simulink model "normal"  (R2020a)
settings: Solver=ode45  StartTime=0.0  StopTime=0.4  FixedStep=1e-6  MaxStep=0.04  RelTol=1e-3  EnableMultiTasking=on
PreLoadFcn:
  | power_13NodeTestFeeder_init;
values from neighbouring files (symbols this model uses):
  C_601 = [1.03835973183e-08  -3.28956213337e-09  -2.07596127216e-09; -3.28956213337e-09  9.8230300863e-09  -1.22250137004e-09; -2.07596127216e-09  -1.22250137004e-09  9.29377945947e-09]    [Finalmat.mat]    (also in bus1.mat; bus10.mat; bus11.mat; bus12.mat)
  C_602 = [9.39333329896e-09  -1.78290377777e-09  -2.78635373607e-09; -1.78290377777e-09  8.5370713848e-09  -1.08586207709e-09; -2.78635373607e-09  -1.08586207709e-09  8.94105559107e-09]    [Finalmat.mat]    (also in bus1.mat; bus10.mat; bus11.mat; bus12.mat)
  C_603 = [0  0  0; 0  7.76272711671e-09  -1.48325331387e-09; 0  -1.48325331387e-09  7.69036927641e-09]    [Finalmat.mat]    (also in bus1.mat; bus10.mat; bus11.mat; bus12.mat)
  C_604 = [7.69036927641e-09  0  -1.48325331387e-09; 0  0  0; -1.48325331387e-09  0  7.76272711671e-09]    [Finalmat.mat]    (also in bus1.mat; bus10.mat; bus11.mat; bus12.mat)
  C_605 = [0  0  0; 0  0  0; 0  0  7.44890176838e-09]    [Finalmat.mat]    (also in bus1.mat; bus10.mat; bus11.mat; bus12.mat)
  C_606 = [1.59697709306e-07  -1.64824237567e-15  -1.64824237567e-15; -1.64824237567e-15  1.59697709306e-07  -1.64824237567e-15; -1.64824237567e-15  -1.64824237567e-15  1.59697709306e-07]    [Finalmat.mat]    (also in bus1.mat; bus10.mat; bus11.mat; bus12.mat)
  C_607 = [1.46679066902e-07  0  0; 0  0  0; 0  0  0]    [Finalmat.mat]    (also in bus1.mat; bus10.mat; bus11.mat; bus12.mat)
  ft2km = 0.0003048    [Finalmat.mat]    (also in bus1.mat; bus10.mat; bus11.mat; bus12.mat)
  L_601 = [0.0016777459142  0.000826923199875  0.000698195470335; 0.000826923199875  0.00172702836123  0.000634408490396; 0.000698195470335  0.000634408490396  0.00170560121035]    [Finalmat.mat]    (also in bus1.mat; bus10.mat; bus11.mat; bus12.mat)
  L_602 = [0.00194723354262  0.000698195470335  0.000826923199875; 0.000698195470335  0.00197508883877  0.000634408490396; 0.000826923199875  0.000634408490396  0.00199635116541]    [Finalmat.mat]    (also in bus1.mat; bus10.mat; bus11.mat; bus12.mat)
  L_603 = [0  0  0; 0  0.00222034730427  0.000756708074671; 0  0.000756708074671  0.00223650007955]    [Finalmat.mat]    (also in bus1.mat; bus10.mat; bus11.mat; bus12.mat)
  L_604 = [0.00223650007955  0  0.000756708074671; 0  0  0; 0.000756708074671  0  0.00222034730427]    [Finalmat.mat]    (also in bus1.mat; bus10.mat; bus11.mat; bus12.mat)
  L_605 = [0  0  0; 0  0  0; 0  0  0.00222100660122]    [Finalmat.mat]    (also in bus1.mat; bus10.mat; bus11.mat; bus12.mat)
  L_606 = [0.000735610572263  5.40623499221e-05  2.35698659721e-05; 5.40623499221e-05  0.000666054744009  5.40623499221e-05; 2.35698659721e-05  5.40623499221e-05  0.000735610572263]    [Finalmat.mat]    (also in bus1.mat; bus10.mat; bus11.mat; bus12.mat)
  L_607 = [0.000844559393295  0  0; 0  0  0; 0  0  0]    [Finalmat.mat]    (also in bus1.mat; bus10.mat; bus11.mat; bus12.mat)
  R_601 = [0.215305653249  0.0969341469174  0.0981768923907; 0.0969341469174  0.209713298619  0.0953807150757; 0.0981768923907  0.0953807150757  0.212136652292]    [Finalmat.mat]    (also in bus1.mat; bus10.mat; bus11.mat; bus12.mat)
  R_602 = [0.467645121603  0.0981768923907  0.0969341469174; 0.0981768923907  0.464476120646  0.0953807150757; 0.0969341469174  0.0953807150757  0.462052766973]    [Finalmat.mat]    (also in bus1.mat; bus10.mat; bus11.mat; bus12.mat)
  R_603 = [0  0  0; 0  0.826052916102  0.128375607392; 0  0.128375607392  0.822573228777]    [Finalmat.mat]    (also in bus1.mat; bus10.mat; bus11.mat; bus12.mat)
  R_604 = [0.822573228777  0  0.128375607392; 0  0  0; 0.128375607392  0  0.826052916102]    [Finalmat.mat]    (also in bus1.mat; bus10.mat; bus11.mat; bus12.mat)
  R_605 = [0  0  0; 0  0  0; 0  0  0.825928641555]    [Finalmat.mat]    (also in bus1.mat; bus10.mat; bus11.mat; bus12.mat)
  R_606 = [0.495979718394  0.198342177539  0.177029092672; 0.198342177539  0.49032522649  0.198342177539; 0.177029092672  0.198342177539  0.495979718394]    [Finalmat.mat]    (also in bus1.mat; bus10.mat; bus11.mat; bus12.mat)
  R_607 = [0.834192898952  0  0; 0  0  0; 0  0  0]    [Finalmat.mat]    (also in bus1.mat; bus10.mat; bus11.mat; bus12.mat)
libraries: neural x322, powerlib x54, powerlib_meascontrol x6, simulink x1
(part 5 of 8)

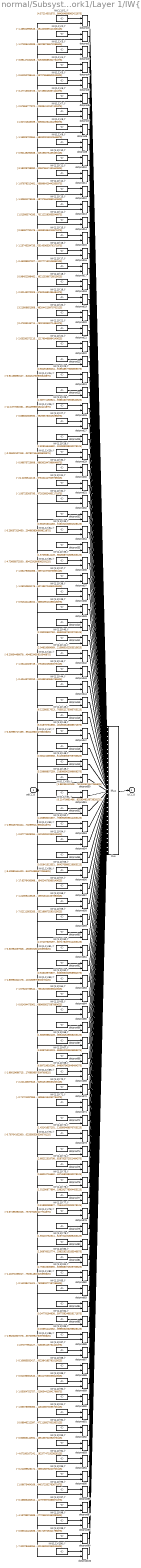
== system normal/Subsystem1/Function Fitting Neural Network1/Layer 1/IW{1,1} ==
  "pd{1,1}" : Inport  PortDimensions=9
      mask Display: e = 0.06;c1 = [120 230 180]/255;c2 = ([120 230 180]+0)/(256+128);c3 = ([120 230 180]+128)/(256+128);patch([0 1 1 0],[0 0 1 1],c1);patch([0 1 1 1-e 1-e 0+e],[0 0 1 1-e 0+e 0+e],c2);patch([0 0 1 1-e 0+e 0+e],[0 1 1 1-e 1-e 0+e],c3);plot([0 1 1 0 0],[0 0 1 1 0]);
  "IW{1,1}(1,:)'" : Constant  Value=[4.57214501575121357035413893754594027996063232421875;1.882606225958038503875968672218732535839080810546875;-5.8020031488986969492316347896121442317962646484375;-1.893288066425211635390724040917120873928070068359375;-0.8587623785139932852672473018174059689044952392578125;4.75157469500696638675663052708841860294342041015625;-8.5282617700155807227702098316513001918792724609375;-3.382695445647363907681892669643275439739227294921875;5.878872822846187062850731308571994304656982421875]
      mask Display: e = 0.06;c1 = [120 150 230]/255;c2 = ([120 150 230]+0)/383;c3 = ([120 150 230]+128)/383;patch([0 1 1 0],[0 0 1 1],c1);patch([0 1 1 1-e 1-e 0+e],[0 0 1 1-e 0+e 0+e],c2);patch([0 0 1 1-e 0+e 0+e],[0 1 1 1-e 1-e 0+e],c3);plot([0 1 1 0 0],[0 0 1 1 0]);disp('Weights');
  "IW{1,1}(10,:)'" : Constant  Value=[-0.901492906386826664544287268654443323612213134765625;-0.113174797714675090531954992911778390407562255859375;1.080394196679439033914604806341230869293212890625;-0.73545756418224861317156637596781365573406219482421875;-0.5017931218574249729869052316644228994846343994140625;-1.384370210252817923191059890086762607097625732421875;0.142477760614644177739052111064665950834751129150390625;0.047994454507014831790012721057792077772319316864013671875;-1.07906134729644254122149504837580025196075439453125]
      mask Display: e = 0.06;c1 = [120 150 230]/255;c2 = ([120 150 230]+0)/383;c3 = ([120 150 230]+128)/383;patch([0 1 1 0],[0 0 1 1],c1);patch([0 1 1 1-e 1-e 0+e],[0 0 1 1-e 0+e 0+e],c2);patch([0 0 1 1-e 0+e 0+e],[0 1 1 1-e 1-e 0+e],c3);plot([0 1 1 0 0],[0 0 1 1 0]);disp('Weights');
  "IW{1,1}(100,:)'" : Constant  Value=[-7.320784632640833677896807785145938396453857421875;-16.1707657106398841051486670039594173431396484375;7.2803217921115379596130878780968487262725830078125;3.3426274799199280352013374795205891132354736328125;2.874821735640806341649522437364794313907623291015625;4.61847119975394004853797014220617711544036865234375;1.3255014486968230702501614359789527952671051025390625;0.304284782798684094728969284915365278720855712890625;-0.269542146930250636760462157326401211321353912353515625]
      mask Display: e = 0.06;c1 = [120 150 230]/255;c2 = ([120 150 230]+0)/383;c3 = ([120 150 230]+128)/383;patch([0 1 1 0],[0 0 1 1],c1);patch([0 1 1 1-e 1-e 0+e],[0 0 1 1-e 0+e 0+e],c2);patch([0 0 1 1-e 0+e 0+e],[0 1 1 1-e 1-e 0+e],c3);plot([0 1 1 0 0],[0 0 1 1 0]);disp('Weights');
  "IW{1,1}(11,:)'" : Constant  Value=[3.182097989903924339927243636338971555233001708984375;-1.2350123444631406766092140969703905284404754638671875;2.388405963368278595027049959753639996051788330078125;-0.86926885397664677146423173326184041798114776611328125;-1.060735410466756345471139866276644170284271240234375;-0.2099496708397343980312399480681051500141620635986328125;4.97375374438937267740357128786854445934295654296875;0.59049268116716879806205042768851853907108306884765625;1.0899488888556165822052435032674111425876617431640625]
      mask Display: e = 0.06;c1 = [120 150 230]/255;c2 = ([120 150 230]+0)/383;c3 = ([120 150 230]+128)/383;patch([0 1 1 0],[0 0 1 1],c1);patch([0 1 1 1-e 1-e 0+e],[0 0 1 1-e 0+e 0+e],c2);patch([0 0 1 1-e 0+e 0+e],[0 1 1 1-e 1-e 0+e],c3);plot([0 1 1 0 0],[0 0 1 1 0]);disp('Weights');
  "IW{1,1}(12,:)'" : Constant  Value=[-1.8787831248148643137341196052148006856441497802734375;0.8158366697060552841236358290188945829868316650390625;1.8402745283322923253166436552419327199459075927734375;-2.500087171504715488623560304404236376285552978515625;0.6981167220195245715075316184083931148052215576171875;0.68711892811027308614058028979343362152576446533203125;-2.837133552361146282549952957197092473506927490234375;2.6394050270587587903037274372763931751251220703125;2.250006537446691989856617510668002068996429443359375]
      mask Display: e = 0.06;c1 = [120 150 230]/255;c2 = ([120 150 230]+0)/383;c3 = ([120 150 230]+128)/383;patch([0 1 1 0],[0 0 1 1],c1);patch([0 1 1 1-e 1-e 0+e],[0 0 1 1-e 0+e 0+e],c2);patch([0 0 1 1-e 0+e 0+e],[0 1 1 1-e 1-e 0+e],c3);plot([0 1 1 0 0],[0 0 1 1 0]);disp('Weights');
  "IW{1,1}(13,:)'" : Constant  Value=[-1.30581276345382235604120069183409214019775390625;-0.0578981895339648333642657007658272050321102142333984375;-0.200199831873287881212064576175180263817310333251953125;0.32696800181646079597186371756833977997303009033203125;0.51819519715458894904003273040871135890483856201171875;-1.05830517304619053930991867673583328723907470703125;-0.90740435735102398240314869326539337635040283203125;-0.428920341006585770227133025400689803063869476318359375;-0.53095640707807023606079610544838942587375640869140625]
      mask Display: e = 0.06;c1 = [120 150 230]/255;c2 = ([120 150 230]+0)/383;c3 = ([120 150 230]+128)/383;patch([0 1 1 0],[0 0 1 1],c1);patch([0 1 1 1-e 1-e 0+e],[0 0 1 1-e 0+e 0+e],c2);patch([0 0 1 1-e 0+e 0+e],[0 1 1 1-e 1-e 0+e],c3);plot([0 1 1 0 0],[0 0 1 1 0]);disp('Weights');
  "IW{1,1}(14,:)'" : Constant  Value=[1.5158057429565598983600693827611394226551055908203125;-1.53943291617461053277793325833044946193695068359375;1.1719124189160725624248016174533404409885406494140625;0.91568727726024423674289209884591400623321533203125;-0.91349144230285539425295837645535357296466827392578125;0.129574899846442492812315094852237962186336517333984375;1.357529536973298700530676796915940940380096435546875;0.9917911601413254008008379969396628439426422119140625;-0.53992566084737869669396559402230195701122283935546875]
      mask Display: e = 0.06;c1 = [120 150 230]/255;c2 = ([120 150 230]+0)/383;c3 = ([120 150 230]+128)/383;patch([0 1 1 0],[0 0 1 1],c1);patch([0 1 1 1-e 1-e 0+e],[0 0 1 1-e 0+e 0+e],c2);patch([0 0 1 1-e 0+e 0+e],[0 1 1 1-e 1-e 0+e],c3);plot([0 1 1 0 0],[0 0 1 1 0]);disp('Weights');
  "IW{1,1}(15,:)'" : Constant  Value=[0.3636779247682031535049418380367569625377655029296875;0.27580226552316544630372163737774826586246490478515625;0.91847507041818976514235828290111385285854339599609375;0.94676222259045050844150637203711085021495819091796875;1.1914278164934548609465991830802522599697113037109375;1.0862301664903963871466885393601842224597930908203125;-0.313351448219361838898322503155213780701160430908203125;0.480054965682457090991874792962335050106048583984375;-1.0512469187967610206868585009942762553691864013671875]
      mask Display: e = 0.06;c1 = [120 150 230]/255;c2 = ([120 150 230]+0)/383;c3 = ([120 150 230]+128)/383;patch([0 1 1 0],[0 0 1 1],c1);patch([0 1 1 1-e 1-e 0+e],[0 0 1 1-e 0+e 0+e],c2);patch([0 0 1 1-e 0+e 0+e],[0 1 1 1-e 1-e 0+e],c3);plot([0 1 1 0 0],[0 0 1 1 0]);disp('Weights');
  "IW{1,1}(16,:)'" : Constant  Value=[-1.2374533473535482830385490160551853477954864501953125;0.84525543133610880897066408579121343791484832763671875;-1.1637539518642545655069397980696521699428558349609375;0.2051190480644304037216585356873110868036746978759765625;2.659058217179519179040880771935917437076568603515625;0.2220786361148645859930894630451803095638751983642578125;0.256689466162800361548335104089346714317798614501953125;0.32918163162337654714661994148627854883670806884765625;-1.539386232767935069887244026176631450653076171875]
      mask Display: e = 0.06;c1 = [120 150 230]/255;c2 = ([120 150 230]+0)/383;c3 = ([120 150 230]+128)/383;patch([0 1 1 0],[0 0 1 1],c1);patch([0 1 1 1-e 1-e 0+e],[0 0 1 1-e 0+e 0+e],c2);patch([0 0 1 1-e 0+e 0+e],[0 1 1 1-e 1-e 0+e],c3);plot([0 1 1 0 0],[0 0 1 1 0]);disp('Weights');
  "IW{1,1}(17,:)'" : Constant  Value=[-0.4528993702754127159693098292336799204349517822265625;0.2996485110712263644217046021367423236370086669921875;-1.3571742827353954208291497707250528037548065185546875;0.72201368049507952395771326337126083672046661376953125;-0.260676388954095783478948078482062555849552154541015625;-1.7370101028329736347899370230152271687984466552734375;-0.72478751750280301369144808631972409784793853759765625;1.6961692464966287019478841102682054042816162109375;-2.777268542019787123109608728555031120777130126953125]
      mask Display: e = 0.06;c1 = [120 150 230]/255;c2 = ([120 150 230]+0)/383;c3 = ([120 150 230]+128)/383;patch([0 1 1 0],[0 0 1 1],c1);patch([0 1 1 1-e 1-e 0+e],[0 0 1 1-e 0+e 0+e],c2);patch([0 0 1 1-e 0+e 0+e],[0 1 1 1-e 1-e 0+e],c3);plot([0 1 1 0 0],[0 0 1 1 0]);disp('Weights');
  "IW{1,1}(18,:)'" : Constant  Value=[0.984523984828047371564707646030001342296600341796875;0.440886294126075828359034858294762670993804931640625;-0.6759076310964935441205625465954653918743133544921875;-1.289035500093658637155158430687151849269866943359375;-0.7106270365609741457291193000855855643749237060546875;-0.00059208655953670529491217333628583219251595437526702880859375;2.360279246169174616198915828135795891284942626953125;2.289325113655392041067671016207896173000335693359375;0.61338355224400320508948425413109362125396728515625]
      mask Display: e = 0.06;c1 = [120 150 230]/255;c2 = ([120 150 230]+0)/383;c3 = ([120 150 230]+128)/383;patch([0 1 1 0],[0 0 1 1],c1);patch([0 1 1 1-e 1-e 0+e],[0 0 1 1-e 0+e 0+e],c2);patch([0 0 1 1-e 0+e 0+e],[0 1 1 1-e 1-e 0+e],c3);plot([0 1 1 0 0],[0 0 1 1 0]);disp('Weights');
  "IW{1,1}(19,:)'" : Constant  Value=[-2.32143070023364384013575545395724475383758544921875;1.35427998731956922284780375775881111621856689453125;-1.1460257544519387717940617221756838262081146240234375;-0.5807263512829130558401402595336548984050750732421875;1.0079516669472294854159599708509631454944610595703125;-2.12978652832783499349034173064865171909332275390625;0.6223670523531816822782047893269918859004974365234375;-1.4856321514957333551620877187815494835376739501953125;0.04807060918235782354113183600929914973676204681396484375]
      mask Display: e = 0.06;c1 = [120 150 230]/255;c2 = ([120 150 230]+0)/383;c3 = ([120 150 230]+128)/383;patch([0 1 1 0],[0 0 1 1],c1);patch([0 1 1 1-e 1-e 0+e],[0 0 1 1-e 0+e 0+e],c2);patch([0 0 1 1-e 0+e 0+e],[0 1 1 1-e 1-e 0+e],c3);plot([0 1 1 0 0],[0 0 1 1 0]);disp('Weights');
  "IW{1,1}(2,:)'" : Constant  Value=[-1.465049905469430147064713310101069509983062744140625;-0.1874316016641332238723549608039320446550846099853515625;-0.06919763970673868669347683635351131670176982879638671875;-0.57055203810173826806106944786733947694301605224609375;3.1381492483832875706184495356865227222442626953125;-0.874421368308234026045511200209148228168487548828125;1.23739151157753735077449164236895740032196044921875;1.3521956808911073100176736261346377432346343994140625;4.10697081729739910116450118948705494403839111328125]
      mask Display: e = 0.06;c1 = [120 150 230]/255;c2 = ([120 150 230]+0)/383;c3 = ([120 150 230]+128)/383;patch([0 1 1 0],[0 0 1 1],c1);patch([0 1 1 1-e 1-e 0+e],[0 0 1 1-e 0+e 0+e],c2);patch([0 0 1 1-e 0+e 0+e],[0 1 1 1-e 1-e 0+e],c3);plot([0 1 1 0 0],[0 0 1 1 0]);disp('Weights');
  "IW{1,1}(20,:)'" : Constant  Value=[3.218086519585205973470465323771350085735321044921875;-16.27590168275634852079747361131012439727783203125;17.987410545814295659283743589185178279876708984375;3.758242055086093547089376443182118237018585205078125;-4.85910970919836326942231607972644269466400146484375;0.3725222076867311660208770263125188648700714111328125;-1.3744616444228034968233487234101630747318267822265625;-5.007581197173916365272816619835793972015380859375;0.24849610765830132397269380817306227982044219970703125]
      mask Display: e = 0.06;c1 = [120 150 230]/255;c2 = ([120 150 230]+0)/383;c3 = ([120 150 230]+128)/383;patch([0 1 1 0],[0 0 1 1],c1);patch([0 1 1 1-e 1-e 0+e],[0 0 1 1-e 0+e 0+e],c2);patch([0 0 1 1-e 0+e 0+e],[0 1 1 1-e 1-e 0+e],c3);plot([0 1 1 0 0],[0 0 1 1 0]);disp('Weights');
  "IW{1,1}(21,:)'" : Constant  Value=[0.47333245711844529335365905353683046996593475341796875;-6.1031253338012145803759267437271773815155029296875;2.142440438103456745722041887347586452960968017578125;2.62530251915655110650504866498522460460662841796875;-1.841367984976616245518243886181153357028961181640625;1.9183672712002162175082276007742621004581451416015625;1.1140395667070130958364870821242220699787139892578125;-0.09091837053477576369164836478375946171581745147705078125;0.8327519583244809009414666434167884290218353271484375]
      mask Display: e = 0.06;c1 = [120 150 230]/255;c2 = ([120 150 230]+0)/383;c3 = ([120 150 230]+128)/383;patch([0 1 1 0],[0 0 1 1],c1);patch([0 1 1 1-e 1-e 0+e],[0 0 1 1-e 0+e 0+e],c2);patch([0 0 1 1-e 0+e 0+e],[0 1 1 1-e 1-e 0+e],c3);plot([0 1 1 0 0],[0 0 1 1 0]);disp('Weights');
  "IW{1,1}(22,:)'" : Constant  Value=[-2.633303721159426569187189670628868043422698974609375;0.2855957397414907728006028264644555747509002685546875;-3.671941916130708083443323630490340292453765869140625;-0.70809683746574425544650921438005752861499786376953125;-0.83203434928004094128795031792833469808101654052734375;0.21652040710604414375239912260440178215503692626953125;-0.6855160542714191507229770650155842304229736328125;-0.77678134128400044833284709966392256319522857666015625;-0.465629395082590991084003917421796359121799468994140625]
      mask Display: e = 0.06;c1 = [120 150 230]/255;c2 = ([120 150 230]+0)/383;c3 = ([120 150 230]+128)/383;patch([0 1 1 0],[0 0 1 1],c1);patch([0 1 1 1-e 1-e 0+e],[0 0 1 1-e 0+e 0+e],c2);patch([0 0 1 1-e 0+e 0+e],[0 1 1 1-e 1-e 0+e],c3);plot([0 1 1 0 0],[0 0 1 1 0]);disp('Weights');
  "IW{1,1}(23,:)'" : Constant  Value=[0.56491806234007679865527506990474648773670196533203125;0.77026935261504358987139085002127103507518768310546875;-0.064774393859191981004386207132483832538127899169921875;1.849415015758316460647847634390927851200103759765625;0.96274697549558718723261563354753889143466949462890625;-1.1368993403818092868817757334909401834011077880859375;0.86488128146804121865187653384055010974407196044921875;0.351346425363474157421705967863090336322784423828125;-0.425453238706487935072431127991876564919948577880859375]
      mask Display: e = 0.06;c1 = [120 150 230]/255;c2 = ([120 150 230]+0)/383;c3 = ([120 150 230]+128)/383;patch([0 1 1 0],[0 0 1 1],c1);patch([0 1 1 1-e 1-e 0+e],[0 0 1 1-e 0+e 0+e],c2);patch([0 0 1 1-e 0+e 0+e],[0 1 1 1-e 1-e 0+e],c3);plot([0 1 1 0 0],[0 0 1 1 0]);disp('Weights');
  "IW{1,1}(24,:)'" : Constant  Value=[-0.91138890127663374496336246011196635663509368896484375;15.0789832454367029868080862797796726226806640625;10.556078107952632905153222964145243167877197265625;-0.9792542115477893549524424088303931057453155517578125;3.0303379951251638857456782716326415538787841796875;-2.761581601481574832490650805993936955928802490234375;-8.3770890674707967349377213395200669765472412109375;-2.070123180109808114224279051995836198329925537109375;-13.6068544965806932367513581993989646434783935546875]
      mask Display: e = 0.06;c1 = [120 150 230]/255;c2 = ([120 150 230]+0)/383;c3 = ([120 150 230]+128)/383;patch([0 1 1 0],[0 0 1 1],c1);patch([0 1 1 1-e 1-e 0+e],[0 0 1 1-e 0+e 0+e],c2);patch([0 0 1 1-e 0+e 0+e],[0 1 1 1-e 1-e 0+e],c3);plot([0 1 1 0 0],[0 0 1 1 0]);disp('Weights');
  "IW{1,1}(25,:)'" : Constant  Value=[2.38771156921450966592601616866886615753173828125;-2.191485976358347187442632275633513927459716796875;3.00359378776327989868377699167467653751373291015625;-0.23173797831026388127639847880345769226551055908203125;-0.99380085545549778913709815242327749729156494140625;0.36246471125366774845844020092044956982135772705078125;2.794875124789037545980363574926741421222686767578125;-0.1950511468235609502386296298936940729618072509765625;-2.01187767968755171210659682401455938816070556640625]
      mask Display: e = 0.06;c1 = [120 150 230]/255;c2 = ([120 150 230]+0)/383;c3 = ([120 150 230]+128)/383;patch([0 1 1 0],[0 0 1 1],c1);patch([0 1 1 1-e 1-e 0+e],[0 0 1 1-e 0+e 0+e],c2);patch([0 0 1 1-e 0+e 0+e],[0 1 1 1-e 1-e 0+e],c3);plot([0 1 1 0 0],[0 0 1 1 0]);disp('Weights');
  "IW{1,1}(26,:)'" : Constant  Value=[-12.1377651561355168752243116614408791065216064453125;8.1591652697612939704185919254086911678314208984375;-3.80045548821983825149573021917603909969329833984375;-2.145339820153546295244950670166872441768646240234375;-3.71648549095900992966789999627508223056793212890625;6.57426106015730749021486190031282603740692138671875;4.48441260631393134872269001789391040802001953125;3.304872366104713687917637798818759620189666748046875;0.8970116797606457748059938239748589694499969482421875]
      mask Display: e = 0.06;c1 = [120 150 230]/255;c2 = ([120 150 230]+0)/383;c3 = ([120 150 230]+128)/383;patch([0 1 1 0],[0 0 1 1],c1);patch([0 1 1 1-e 1-e 0+e],[0 0 1 1-e 0+e 0+e],c2);patch([0 0 1 1-e 0+e 0+e],[0 1 1 1-e 1-e 0+e],c3);plot([0 1 1 0 0],[0 0 1 1 0]);disp('Weights');
  "IW{1,1}(27,:)'" : Constant  Value=[-0.88832363930812319186003378490568138659000396728515625;0.42785830611103670140238364183460362255573272705078125;0.80867323101893229253533945666276849806308746337890625;-0.77923766081130063643200855949544347822666168212890625;-0.56145456173519547871109125480870716273784637451171875;-0.60230053309847331188819907765719108283519744873046875;-1.3050830682250218472972846939228475093841552734375;-0.806330916403047215368360411957837641239166259765625;-0.441184745456177640487993585338699631392955780029296875]
      mask Display: e = 0.06;c1 = [120 150 230]/255;c2 = ([120 150 230]+0)/383;c3 = ([120 150 230]+128)/383;patch([0 1 1 0],[0 0 1 1],c1);patch([0 1 1 1-e 1-e 0+e],[0 0 1 1-e 0+e 0+e],c2);patch([0 0 1 1-e 0+e 0+e],[0 1 1 1-e 1-e 0+e],c3);plot([0 1 1 0 0],[0 0 1 1 0]);disp('Weights');
  "IW{1,1}(28,:)'" : Constant  Value=[2.82816646582525788033990465919487178325653076171875;0.35954363621026186326190554609638638794422149658203125;1.632878770180271832401786014088429510593414306640625;-0.0101763750096381978826887149125468567945063114166259765625;-1.059871357865847851797980183619074523448944091796875;-1.537916378610710399499339473550207912921905517578125;-0.316755007210310746135206727558397687971591949462890625;0.01847910556224353906262791724657290615141391754150390625;-2.461970474843802936248948753927834331989288330078125]
      mask Display: e = 0.06;c1 = [120 150 230]/255;c2 = ([120 150 230]+0)/383;c3 = ([120 150 230]+128)/383;patch([0 1 1 0],[0 0 1 1],c1);patch([0 1 1 1-e 1-e 0+e],[0 0 1 1-e 0+e 0+e],c2);patch([0 0 1 1-e 0+e 0+e],[0 1 1 1-e 1-e 0+e],c3);plot([0 1 1 0 0],[0 0 1 1 0]);disp('Weights');
  "IW{1,1}(29,:)'" : Constant  Value=[-0.2562310731830372834139097903971560299396514892578125;-0.026650997824419812853857791878908756189048290252685546875;0.5146222044853010491038958207354880869388580322265625;-0.08863109829785020821191210416145622730255126953125;1.0860301622782368990982604373130016028881072998046875;-0.83558626518929435267324379310593940317630767822265625;0.75271604021013638341486284843995235860347747802734375;-1.5471971637303971736088215038762427866458892822265625;-1.534789360688019854705999023281037807464599609375]
      mask Display: e = 0.06;c1 = [120 150 230]/255;c2 = ([120 150 230]+0)/383;c3 = ([120 150 230]+128)/383;patch([0 1 1 0],[0 0 1 1],c1);patch([0 1 1 1-e 1-e 0+e],[0 0 1 1-e 0+e 0+e],c2);patch([0 0 1 1-e 0+e 0+e],[0 1 1 1-e 1-e 0+e],c3);plot([0 1 1 0 0],[0 0 1 1 0]);disp('Weights');
  "IW{1,1}(3,:)'" : Constant  Value=[-1.273064109391197629150838110945187509059906005859375;-0.1746139127475550001378223896608687937259674072265625;-1.97988528255410134448766257264651358127593994140625;2.115356814135119112307847899501211941242218017578125;3.676111139990880349870394638855941593647003173828125;-0.634748668186627451603953886660747230052947998046875;-2.02947200057094079284070176072418689727783203125;0.70475348178681518351851309489575214684009552001953125;4.35348031629683962506760508404113352298736572265625]
      mask Display: e = 0.06;c1 = [120 150 230]/255;c2 = ([120 150 230]+0)/383;c3 = ([120 150 230]+128)/383;patch([0 1 1 0],[0 0 1 1],c1);patch([0 1 1 1-e 1-e 0+e],[0 0 1 1-e 0+e 0+e],c2);patch([0 0 1 1-e 0+e 0+e],[0 1 1 1-e 1-e 0+e],c3);plot([0 1 1 0 0],[0 0 1 1 0]);disp('Weights');
  "IW{1,1}(30,:)'" : Constant  Value=[-0.9987572360844405583435445805662311613559722900390625;-0.298860431335690790444203912556986324489116668701171875;-1.0756527117942642490788784925825893878936767578125;-0.2325361948543681334111710157230845652520656585693359375;-0.97740459386404177077878330237581394612789154052734375;0.1938044318657854148124641824324498884379863739013671875;0.8947266366516830604638244039961136877536773681640625;-0.6522406157472897536564460096997208893299102783203125;-1.1122828714271715266903584051760844886302947998046875]
      mask Display: e = 0.06;c1 = [120 150 230]/255;c2 = ([120 150 230]+0)/383;c3 = ([120 150 230]+128)/383;patch([0 1 1 0],[0 0 1 1],c1);patch([0 1 1 1-e 1-e 0+e],[0 0 1 1-e 0+e 0+e],c2);patch([0 0 1 1-e 0+e 0+e],[0 1 1 1-e 1-e 0+e],c3);plot([0 1 1 0 0],[0 0 1 1 0]);disp('Weights');
  "IW{1,1}(31,:)'" : Constant  Value=[-21.2230544116653589981069671921432018280029296875;17.38640835398523876165199908427894115447998046875;4.29589166719302806285440965439192950725555419921875;1.18972370473984323524518913473002612590789794921875;-1.649465861026556012802757322788238525390625;-1.4940892099984635077447592266253195703029632568359375;1.65452073013394596046055085025727748870849609375;-7.5067697997629547757014734088443219661712646484375;6.34941966304106841789689497090876102447509765625]
      mask Display: e = 0.06;c1 = [120 150 230]/255;c2 = ([120 150 230]+0)/383;c3 = ([120 150 230]+128)/383;patch([0 1 1 0],[0 0 1 1],c1);patch([0 1 1 1-e 1-e 0+e],[0 0 1 1-e 0+e 0+e],c2);patch([0 0 1 1-e 0+e 0+e],[0 1 1 1-e 1-e 0+e],c3);plot([0 1 1 0 0],[0 0 1 1 0]);disp('Weights');
  "IW{1,1}(32,:)'" : Constant  Value=[-1.9372530579534597006130525187472812831401824951171875;-0.034387366226837280669403895672076032496988773345947265625;-1.8460191297376915553485332566197030246257781982421875;-1.1491734164584344046744490697165019810199737548828125;-1.0773258382449684145143464775173924863338470458984375;0.5971848864048723282138553258846513926982879638671875;-1.0895137852805845124493089315365068614482879638671875;0.5721940530226146126580033524078316986560821533203125;-0.84712647433286036857680301181972026824951171875]
      mask Display: e = 0.06;c1 = [120 150 230]/255;c2 = ([120 150 230]+0)/383;c3 = ([120 150 230]+128)/383;patch([0 1 1 0],[0 0 1 1],c1);patch([0 1 1 1-e 1-e 0+e],[0 0 1 1-e 0+e 0+e],c2);patch([0 0 1 1-e 0+e 0+e],[0 1 1 1-e 1-e 0+e],c3);plot([0 1 1 0 0],[0 0 1 1 0]);disp('Weights');
  "IW{1,1}(33,:)'" : Constant  Value=[0.6529160448325892485144095189752988517284393310546875;-1.0012486019936506220773253517108969390392303466796875;0.404005214638427478934801229115691967308521270751953125;-0.08869602104426006772275314915532362647354602813720703125;1.5234337610562678211323373034247197210788726806640625;-0.0296601631566312147481045968788748723454773426055908203125;1.578527371192719019887817921699024736881256103515625;-0.483526252419098245827200344137963838875293731689453125;2.691032424683868828907407078077085316181182861328125]
      mask Display: e = 0.06;c1 = [120 150 230]/255;c2 = ([120 150 230]+0)/383;c3 = ([120 150 230]+128)/383;patch([0 1 1 0],[0 0 1 1],c1);patch([0 1 1 1-e 1-e 0+e],[0 0 1 1-e 0+e 0+e],c2);patch([0 0 1 1-e 0+e 0+e],[0 1 1 1-e 1-e 0+e],c3);plot([0 1 1 0 0],[0 0 1 1 0]);disp('Weights');
  "IW{1,1}(34,:)'" : Constant  Value=[-0.280373194502217704116020513538387604057788848876953125;-2.8648874605944225635312250233255326747894287109375;0.13981534693347297260146433472982607781887054443359375;-0.87154104232599227675137854021159000694751739501953125;0.59615182479228423506611989068915136158466339111328125;1.1000011216169645056339732036576606333255767822265625;-1.551372378155303710656198745709843933582305908203125;-2.730637946961703921289199570310302078723907470703125;-0.96224054502257139187548773406888358294963836669921875]
      mask Display: e = 0.06;c1 = [120 150 230]/255;c2 = ([120 150 230]+0)/383;c3 = ([120 150 230]+128)/383;patch([0 1 1 0],[0 0 1 1],c1);patch([0 1 1 1-e 1-e 0+e],[0 0 1 1-e 0+e 0+e],c2);patch([0 0 1 1-e 0+e 0+e],[0 1 1 1-e 1-e 0+e],c3);plot([0 1 1 0 0],[0 0 1 1 0]);disp('Weights');
  "IW{1,1}(35,:)'" : Constant  Value=[1.5709081414954437772024675723514519631862640380859375;-4.22386531174724577653023516177199780941009521484375;3.332881064917796010149686480872333049774169921875;-0.78210339536838191509815487734158523380756378173828125;0.43417624969241419563559247762896120548248291015625;1.200110893873937545350827349466271698474884033203125;-0.65289554267587568414654697335208766162395477294921875;5.60910565954152229295459619606845080852508544921875;-6.69035045844220821464887194451875984668731689453125]
      mask Display: e = 0.06;c1 = [120 150 230]/255;c2 = ([120 150 230]+0)/383;c3 = ([120 150 230]+128)/383;patch([0 1 1 0],[0 0 1 1],c1);patch([0 1 1 1-e 1-e 0+e],[0 0 1 1-e 0+e 0+e],c2);patch([0 0 1 1-e 0+e 0+e],[0 1 1 1-e 1-e 0+e],c3);plot([0 1 1 0 0],[0 0 1 1 0]);disp('Weights');
  "IW{1,1}(36,:)'" : Constant  Value=[-4.73608573200478932818668909021653234958648681640625;3.259068429729173654862961484468542039394378662109375;1.870367688521361149156518877134658396244049072265625;-3.9085077606485043588691041804850101470947265625;-0.132532681312490241420931624816148541867733001708984375;1.07321546901653075423155314638279378414154052734375;3.14899895426178577650944134802557528018951416015625;-1.0490359730371248137004158706986345350742340087890625;-5.4847780930769847174133246880955994129180908203125]
      mask Display: e = 0.06;c1 = [120 150 230]/255;c2 = ([120 150 230]+0)/383;c3 = ([120 150 230]+128)/383;patch([0 1 1 0],[0 0 1 1],c1);patch([0 1 1 1-e 1-e 0+e],[0 0 1 1-e 0+e 0+e],c2);patch([0 0 1 1-e 0+e 0+e],[0 1 1 1-e 1-e 0+e],c3);plot([0 1 1 0 0],[0 0 1 1 0]);disp('Weights');
  "IW{1,1}(37,:)'" : Constant  Value=[-1.6547906206673328455281080096028745174407958984375;-3.792463282037272787050596889457665383815765380859375;1.022480990224386321330030114040710031986236572265625;-1.41514034474598560109370737336575984954833984375;-0.0481143329803337127525963978769141249358654022216796875;-0.61324450181596523723470681943581439554691314697265625;-1.3073911340950215009826251844060607254505157470703125;-0.6260849341527563449716353716212324798107147216796875;-0.84798662852783213139673534897156059741973876953125]
      mask Display: e = 0.06;c1 = [120 150 230]/255;c2 = ([120 150 230]+0)/383;c3 = ([120 150 230]+128)/383;patch([0 1 1 0],[0 0 1 1],c1);patch([0 1 1 1-e 1-e 0+e],[0 0 1 1-e 0+e 0+e],c2);patch([0 0 1 1-e 0+e 0+e],[0 1 1 1-e 1-e 0+e],c3);plot([0 1 1 0 0],[0 0 1 1 0]);disp('Weights');
  "IW{1,1}(38,:)'" : Constant  Value=[-1.260105811766427219566821804619394242763519287109375;-0.86726445474906288524152842001058161258697509765625;4.4408342530586164542683036415837705135345458984375;5.05462080690503956503789595444686710834503173828125;-0.7458114846798424846241459817974828183650970458984375;-0.385168955880710262018595813060528598725795745849609375;-3.5337239758800560451845740317367017269134521484375;-4.59283664819310377680494639207608997821807861328125;-0.554578244091102678936522352159954607486724853515625]
      mask Display: e = 0.06;c1 = [120 150 230]/255;c2 = ([120 150 230]+0)/383;c3 = ([120 150 230]+128)/383;patch([0 1 1 0],[0 0 1 1],c1);patch([0 1 1 1-e 1-e 0+e],[0 0 1 1-e 0+e 0+e],c2);patch([0 0 1 1-e 0+e 0+e],[0 1 1 1-e 1-e 0+e],c3);plot([0 1 1 0 0],[0 0 1 1 0]);disp('Weights');
  "IW{1,1}(39,:)'" : Constant  Value=[-0.91342448152657784721242251180228777229785919189453125;-0.2276880613276453801940846233264892362058162689208984375;0.216120568324401018944769248264492489397525787353515625;0.279050464407995857385458293720148503780364990234375;-1.2470189329715950510291122554917819797992706298828125;-0.1573403547029812443724949844181537628173828125;-2.848487435814683887969067654921673238277435302734375;-1.501075399926252718074692893424071371555328369140625;-0.3034357923850758975703456599148921668529510498046875]
      mask Display: e = 0.06;c1 = [120 150 230]/255;c2 = ([120 150 230]+0)/383;c3 = ([120 150 230]+128)/383;patch([0 1 1 0],[0 0 1 1],c1);patch([0 1 1 1-e 1-e 0+e],[0 0 1 1-e 0+e 0+e],c2);patch([0 0 1 1-e 0+e 0+e],[0 1 1 1-e 1-e 0+e],c3);plot([0 1 1 0 0],[0 0 1 1 0]);disp('Weights');
  "IW{1,1}(4,:)'" : Constant  Value=[-3.89147184328426920529864219133742153644561767578125;3.459343926073256358932894727331586182117462158203125;-3.901582530636779733157482041860930621623992919921875;-1.2529766928303931461385900547611527144908905029296875;1.2930662567929680495382172011886723339557647705078125;-1.4188815690276730396846005533006973564624786376953125;3.30385499606749188927778959623537957668304443359375;4.30601828701230271434496899018995463848114013671875;-2.019042118362074145210272035910747945308685302734375]
      mask Display: e = 0.06;c1 = [120 150 230]/255;c2 = ([120 150 230]+0)/383;c3 = ([120 150 230]+128)/383;patch([0 1 1 0],[0 0 1 1],c1);patch([0 1 1 1-e 1-e 0+e],[0 0 1 1-e 0+e 0+e],c2);patch([0 0 1 1-e 0+e 0+e],[0 1 1 1-e 1-e 0+e],c3);plot([0 1 1 0 0],[0 0 1 1 0]);disp('Weights');
  "IW{1,1}(40,:)'" : Constant  Value=[2.280006327502011487240451970137655735015869140625;-2.960340871458381428737993701361119747161865234375;3.710286991107662135647160539519973099231719970703125;1.7881861683726614220546480282791890203952789306640625;-1.21956172031550824641499275458045303821563720703125;-0.61482727497653610893024733741185627877712249755859375;-3.215466035704943603690253439708612859249114990234375;0.390531736822932351582693399905110709369182586669921875;0.485190019842106690095562271380913443863391876220703125]
      mask Display: e = 0.06;c1 = [120 150 230]/255;c2 = ([120 150 230]+0)/383;c3 = ([120 150 230]+128)/383;patch([0 1 1 0],[0 0 1 1],c1);patch([0 1 1 1-e 1-e 0+e],[0 0 1 1-e 0+e 0+e],c2);patch([0 0 1 1-e 0+e 0+e],[0 1 1 1-e 1-e 0+e],c3);plot([0 1 1 0 0],[0 0 1 1 0]);disp('Weights');
  "IW{1,1}(41,:)'" : Constant  Value=[2.0481956906964580156227384577505290508270263671875;0.859554384584698905058530726819299161434173583984375;2.725886455265848606899226069799624383449554443359375;0.2260825309211777212059502062402316369116306304931640625;-0.82525102251196147395972957383492030203342437744140625;0.743435449833508510408819347503595054149627685546875;1.0238058376692169559873946127481758594512939453125;0.354984915450379967527538838112377561628818511962890625;-0.407063535495426676025232382016838528215885162353515625]
      mask Display: e = 0.06;c1 = [120 150 230]/255;c2 = ([120 150 230]+0)/383;c3 = ([120 150 230]+128)/383;patch([0 1 1 0],[0 0 1 1],c1);patch([0 1 1 1-e 1-e 0+e],[0 0 1 1-e 0+e 0+e],c2);patch([0 0 1 1-e 0+e 0+e],[0 1 1 1-e 1-e 0+e],c3);plot([0 1 1 0 0],[0 0 1 1 0]);disp('Weights');
  "IW{1,1}(42,:)'" : Constant  Value=[-6.2093446667831297958173308870755136013031005859375;-7.79394615880087204828896574326790869235992431640625;-0.233526348447979315015032852898002602159976959228515625;3.78428251311718089056057579000480473041534423828125;1.514861585424735590521549966069869697093963623046875;3.648175482940148928179269205429591238498687744140625;4.27427579049037742464633993222378194332122802734375;3.12509590011777493856470755417831242084503173828125;-1.145192992502511497576733745518140494823455810546875]
      mask Display: e = 0.06;c1 = [120 150 230]/255;c2 = ([120 150 230]+0)/383;c3 = ([120 150 230]+128)/383;patch([0 1 1 0],[0 0 1 1],c1);patch([0 1 1 1-e 1-e 0+e],[0 0 1 1-e 0+e 0+e],c2);patch([0 0 1 1-e 0+e 0+e],[0 1 1 1-e 1-e 0+e],c3);plot([0 1 1 0 0],[0 0 1 1 0]);disp('Weights');
  "IW{1,1}(43,:)'" : Constant  Value=[-1.33442026749275033381536559318192303180694580078125;-1.612620029591127046586507276515476405620574951171875;-0.34146945435227415988066468344186432659626007080078125;2.5259282671398981534593985998071730136871337890625;0.75062032032171488449279195265262387692928314208984375;3.183842110728863250557196806767024099826812744140625;3.505507379330950801232802405138500034809112548828125;2.21396331769093723806918205809779465198516845703125;5.14033135835540111457930834149010479450225830078125]
      mask Display: e = 0.06;c1 = [120 150 230]/255;c2 = ([120 150 230]+0)/383;c3 = ([120 150 230]+128)/383;patch([0 1 1 0],[0 0 1 1],c1);patch([0 1 1 1-e 1-e 0+e],[0 0 1 1-e 0+e 0+e],c2);patch([0 0 1 1-e 0+e 0+e],[0 1 1 1-e 1-e 0+e],c3);plot([0 1 1 0 0],[0 0 1 1 0]);disp('Weights');
  "IW{1,1}(44,:)'" : Constant  Value=[-0.404437320102107644714806156116537749767303466796875;-0.89483480675924198521897778846323490142822265625;-0.36393634805201580117994808460935018956661224365234375;-0.80784461164074772288046233370550908148288726806640625;-1.319887663125455024015764138312079012393951416015625;-0.517405527398214104550788761116564273834228515625;-2.619917563217764477911941867205314338207244873046875;-0.65019839853435268395287494058720767498016357421875;-5.38242466892981585857569371000863611698150634765625]
      mask Display: e = 0.06;c1 = [120 150 230]/255;c2 = ([120 150 230]+0)/383;c3 = ([120 150 230]+128)/383;patch([0 1 1 0],[0 0 1 1],c1);patch([0 1 1 1-e 1-e 0+e],[0 0 1 1-e 0+e 0+e],c2);patch([0 0 1 1-e 0+e 0+e],[0 1 1 1-e 1-e 0+e],c3);plot([0 1 1 0 0],[0 0 1 1 0]);disp('Weights');
  "IW{1,1}(45,:)'" : Constant  Value=[6.12288317013641947283986155525781214237213134765625;10.6304077127000482505536638200283050537109375;16.828317110034088699421772616915404796600341796875;0.480006240364688363531087134106201119720935821533203125;-3.030836669137740191359853270114399492740631103515625;-6.999151186851662487242720089852809906005859375;-5.9702070757160310421340909670107066631317138671875;-4.3988675496288056621096984599716961383819580078125;-4.68065715024235107222239093971438705921173095703125]
      mask Display: e = 0.06;c1 = [120 150 230]/255;c2 = ([120 150 230]+0)/383;c3 = ([120 150 230]+128)/383;patch([0 1 1 0],[0 0 1 1],c1);patch([0 1 1 1-e 1-e 0+e],[0 0 1 1-e 0+e 0+e],c2);patch([0 0 1 1-e 0+e 0+e],[0 1 1 1-e 1-e 0+e],c3);plot([0 1 1 0 0],[0 0 1 1 0]);disp('Weights');
  "IW{1,1}(46,:)'" : Constant  Value=[6.31876781866938141973832898656837642192840576171875;6.92142631840081978822354358271695673465728759765625;-1.4815980459966937576865575465490110218524932861328125;4.0282385737923771529267469304613769054412841796875;-6.65040267508876592472688571433536708354949951171875;-4.6374232261565975221628832514397799968719482421875;7.71793169818121338465743974666111171245574951171875;-9.2465905551999956202280372963286936283111572265625;1.4061648337785441764680172127555124461650848388671875]
      mask Display: e = 0.06;c1 = [120 150 230]/255;c2 = ([120 150 230]+0)/383;c3 = ([120 150 230]+128)/383;patch([0 1 1 0],[0 0 1 1],c1);patch([0 1 1 1-e 1-e 0+e],[0 0 1 1-e 0+e 0+e],c2);patch([0 0 1 1-e 0+e 0+e],[0 1 1 1-e 1-e 0+e],c3);plot([0 1 1 0 0],[0 0 1 1 0]);disp('Weights');
  "IW{1,1}(47,:)'" : Constant  Value=[-0.329967174590527989597177338509936816990375518798828125;-0.809733955019600326608042450970970094203948974609375;0.0996942410880331808531451542876311577856540679931640625;-1.5857211906671355716724747253465466201305389404296875;-1.778677732315499415705062347115017473697662353515625;-0.166669253940795403234886862264829687774181365966796875;0.61014363055744713637551512874779291450977325439453125;-1.1294365329561146804593363413005135953426361083984375;-0.21039033829284026211325908661819994449615478515625]
      mask Display: e = 0.06;c1 = [120 150 230]/255;c2 = ([120 150 230]+0)/383;c3 = ([120 150 230]+128)/383;patch([0 1 1 0],[0 0 1 1],c1);patch([0 1 1 1-e 1-e 0+e],[0 0 1 1-e 0+e 0+e],c2);patch([0 0 1 1-e 0+e 0+e],[0 1 1 1-e 1-e 0+e],c3);plot([0 1 1 0 0],[0 0 1 1 0]);disp('Weights');
  "IW{1,1}(48,:)'" : Constant  Value=[0.381210893685120344454020369084901176393032073974609375;-3.127481883483996139005967052071355283260345458984375;-5.8870451205807459160723738023079931735992431640625;0.9112040794954452405107758750091306865215301513671875;0.78202325166951125456904492239118553698062896728515625;0.5468323643589607652160111683770082890987396240234375;3.082137085986965896466927006258629262447357177734375;3.48581097620395841119034230359829962253570556640625;1.771530961345254784333747011260129511356353759765625]
      mask Display: e = 0.06;c1 = [120 150 230]/255;c2 = ([120 150 230]+0)/383;c3 = ([120 150 230]+128)/383;patch([0 1 1 0],[0 0 1 1],c1);patch([0 1 1 1-e 1-e 0+e],[0 0 1 1-e 0+e 0+e],c2);patch([0 0 1 1-e 0+e 0+e],[0 1 1 1-e 1-e 0+e],c3);plot([0 1 1 0 0],[0 0 1 1 0]);disp('Weights');
  "IW{1,1}(49,:)'" : Constant  Value=[5.33968807259485789273867339943535625934600830078125;-1.0478549921619750850965147037641145288944244384765625;1.8039010477897032824756706759217195212841033935546875;-0.71470670968520322308137338040978647768497467041015625;-1.4161887788315741243394541015732102096080780029296875;3.0905944704859269478447458823211491107940673828125;-0.1592048854974729976685665633340249769389629364013671875;-0.300933133992199619566321189267910085618495941162109375;-6.617107841635853304751435643993318080902099609375]
      mask Display: e = 0.06;c1 = [120 150 230]/255;c2 = ([120 150 230]+0)/383;c3 = ([120 150 230]+128)/383;patch([0 1 1 0],[0 0 1 1],c1);patch([0 1 1 1-e 1-e 0+e],[0 0 1 1-e 0+e 0+e],c2);patch([0 0 1 1-e 0+e 0+e],[0 1 1 1-e 1-e 0+e],c3);plot([0 1 1 0 0],[0 0 1 1 0]);disp('Weights');
  "IW{1,1}(5,:)'" : Constant  Value=[-0.612527864443540348560190977877937257289886474609375;2.63701056377172360356553326710127294063568115234375;-0.2344164921880433072320926157772191800177097320556640625;3.326451066418935287316571702831424772739410400390625;-0.3574935045143234901843243278563022613525390625;2.6130973580464154082392269629053771495819091796875;0.3735527265671871877117382609867490828037261962890625;0.04584050982560851361657938696225755847990512847900390625;-1.2960501074079913141900988193810917437076568603515625]
      mask Display: e = 0.06;c1 = [120 150 230]/255;c2 = ([120 150 230]+0)/383;c3 = ([120 150 230]+128)/383;patch([0 1 1 0],[0 0 1 1],c1);patch([0 1 1 1-e 1-e 0+e],[0 0 1 1-e 0+e 0+e],c2);patch([0 0 1 1-e 0+e 0+e],[0 1 1 1-e 1-e 0+e],c3);plot([0 1 1 0 0],[0 0 1 1 0]);disp('Weights');
  "IW{1,1}(50,:)'" : Constant  Value=[1.8823841250808204250688504544086754322052001953125;1.0559600434175007155346293075126595795154571533203125;-3.165147826004930831089723142213188111782073974609375;-1.7056780252132259789732415811158716678619384765625;-0.08936033812179748625492692326588439755141735076904296875;-0.75117755693723997634236866360879503190517425537109375;1.05783644150837830011369078420102596282958984375;0.9932055831634831744025859734392724931240081787109375;0.255838182476943620802245504819438792765140533447265625]
      mask Display: e = 0.06;c1 = [120 150 230]/255;c2 = ([120 150 230]+0)/383;c3 = ([120 150 230]+128)/383;patch([0 1 1 0],[0 0 1 1],c1);patch([0 1 1 1-e 1-e 0+e],[0 0 1 1-e 0+e 0+e],c2);patch([0 0 1 1-e 0+e 0+e],[0 1 1 1-e 1-e 0+e],c3);plot([0 1 1 0 0],[0 0 1 1 0]);disp('Weights');
  "IW{1,1}(51,:)'" : Constant  Value=[0.214708614668400077363230593618936836719512939453125;-0.5401148895579357400720255100168287754058837890625;-1.0797109284227470737960175029002130031585693359375;1.016140436607881891717397593311034142971038818359375;-0.89509991282290091163531542406417429447174072265625;0.9768085213100976549327469911077059805393218994140625;-0.427687062935336259617002951927133835852146148681640625;0.98359039993476127250460194773040711879730224609375;1.4053241377302569947715937814791686832904815673828125]
      mask Display: e = 0.06;c1 = [120 150 230]/255;c2 = ([120 150 230]+0)/383;c3 = ([120 150 230]+128)/383;patch([0 1 1 0],[0 0 1 1],c1);patch([0 1 1 1-e 1-e 0+e],[0 0 1 1-e 0+e 0+e],c2);patch([0 0 1 1-e 0+e 0+e],[0 1 1 1-e 1-e 0+e],c3);plot([0 1 1 0 0],[0 0 1 1 0]);disp('Weights');
  "IW{1,1}(52,:)'" : Constant  Value=[4.2685800163762284142876524128951132297515869140625;4.98140587263257206274147392832674086093902587890625;-12.515494125378463508013737737201154232025146484375;6.8333700814316298277617534040473401546478271484375;0.347782224903877057453627230643178336322307586669921875;0.53856720311356098829236316305468790233135223388671875;-2.86049323039552039205091205076314508914947509765625;-2.2895714722593307755005298531614243984222412109375;2.376065876767160744975626585073769092559814453125]
      mask Display: e = 0.06;c1 = [120 150 230]/255;c2 = ([120 150 230]+0)/383;c3 = ([120 150 230]+128)/383;patch([0 1 1 0],[0 0 1 1],c1);patch([0 1 1 1-e 1-e 0+e],[0 0 1 1-e 0+e 0+e],c2);patch([0 0 1 1-e 0+e 0+e],[0 1 1 1-e 1-e 0+e],c3);plot([0 1 1 0 0],[0 0 1 1 0]);disp('Weights');
  "IW{1,1}(53,:)'" : Constant  Value=[-1.9554670042478707880917454531299881637096405029296875;1.69625825691849652088194488896988332271575927734375;-1.1970874421376687113394154948764480650424957275390625;1.1117797016042045843420282835722900927066802978515625;-0.90863686513132380095925100249587558209896087646484375;-0.7950237696005302279189663750003091990947723388671875;-1.5604125819920271478480344740091823041439056396484375;-0.9118121519169786193259596984717063605785369873046875;-1.51662784590357002656446638866327702999114990234375]
      mask Display: e = 0.06;c1 = [120 150 230]/255;c2 = ([120 150 230]+0)/383;c3 = ([120 150 230]+128)/383;patch([0 1 1 0],[0 0 1 1],c1);patch([0 1 1 1-e 1-e 0+e],[0 0 1 1-e 0+e 0+e],c2);patch([0 0 1 1-e 0+e 0+e],[0 1 1 1-e 1-e 0+e],c3);plot([0 1 1 0 0],[0 0 1 1 0]);disp('Weights');
  "IW{1,1}(54,:)'" : Constant  Value=[-0.8777150909468287576231659841141663491725921630859375;1.4085336466022873036507689903373830020427703857421875;-0.3457668464967316168667821330018341541290283203125;1.3310392902458383357355842235847376286983489990234375;-0.691831136969676574466348029091022908687591552734375;0.32975466552534993258660733772558160126209259033203125;-1.015329999687038853295462104142643511295318603515625;-2.788840081843814378004253740073181688785552978515625;-0.9619262173108982239000397385098040103912353515625]
      mask Display: e = 0.06;c1 = [120 150 230]/255;c2 = ([120 150 230]+0)/383;c3 = ([120 150 230]+128)/383;patch([0 1 1 0],[0 0 1 1],c1);patch([0 1 1 1-e 1-e 0+e],[0 0 1 1-e 0+e 0+e],c2);patch([0 0 1 1-e 0+e 0+e],[0 1 1 1-e 1-e 0+e],c3);plot([0 1 1 0 0],[0 0 1 1 0]);disp('Weights');
  "IW{1,1}(55,:)'" : Constant  Value=[0.029413133514956717184940515608104760758578777313232421875;2.228019601206797428716299691586755216121673583984375;-0.501039620217258008239014088758267462253570556640625;-1.27968307726629060283585204160772264003753662109375;1.6310048626805293547903374928864650428295135498046875;0.68148364696386531935701214024447835981845855712890625;0.467872711076354363957108262184192426502704620361328125;0.63402980121368301968942660096217878162860870361328125;-0.6139566623606473871888056237366981804370880126953125]
      mask Display: e = 0.06;c1 = [120 150 230]/255;c2 = ([120 150 230]+0)/383;c3 = ([120 150 230]+128)/383;patch([0 1 1 0],[0 0 1 1],c1);patch([0 1 1 1-e 1-e 0+e],[0 0 1 1-e 0+e 0+e],c2);patch([0 0 1 1-e 0+e 0+e],[0 1 1 1-e 1-e 0+e],c3);plot([0 1 1 0 0],[0 0 1 1 0]);disp('Weights');
  "IW{1,1}(56,:)'" : Constant  Value=[-9.4098164442060880929830091190524399280548095703125;-1.192369760387879562557600365835241973400115966796875;12.04764844149713809429158573038876056671142578125;-0.08770055792826129958950076570545206777751445770263671875;-0.95073483772437483718675821364740841090679168701171875;0.84211377318583047202338320857961662113666534423828125;-1.2657798532774495736674680301803164184093475341796875;1.4612978423911051617523071399773471057415008544921875;-3.106973248183868552274589092121459543704986572265625]
      mask Display: e = 0.06;c1 = [120 150 230]/255;c2 = ([120 150 230]+0)/383;c3 = ([120 150 230]+128)/383;patch([0 1 1 0],[0 0 1 1],c1);patch([0 1 1 1-e 1-e 0+e],[0 0 1 1-e 0+e 0+e],c2);patch([0 0 1 1-e 0+e 0+e],[0 1 1 1-e 1-e 0+e],c3);plot([0 1 1 0 0],[0 0 1 1 0]);disp('Weights');
  "IW{1,1}(57,:)'" : Constant  Value=[-17.637643098890539050671577570028603076934814453125;2.125595336689284575726333059719763696193695068359375;9.2343454898093710880857543088495731353759765625;-3.73604521387274957078261650167405605316162109375;-3.12822281016979975021286008995957672595977783203125;-7.28199954443057873021416526171378791332244873046875;19.0367560266428341719802119769155979156494140625;-3.1847001873681417549732941552065312862396240234375;10.391026762005200367866564192809164524078369140625]
      mask Display: e = 0.06;c1 = [120 150 230]/255;c2 = ([120 150 230]+0)/383;c3 = ([120 150 230]+128)/383;patch([0 1 1 0],[0 0 1 1],c1);patch([0 1 1 1-e 1-e 0+e],[0 0 1 1-e 0+e 0+e],c2);patch([0 0 1 1-e 0+e 0+e],[0 1 1 1-e 1-e 0+e],c3);plot([0 1 1 0 0],[0 0 1 1 0]);disp('Weights');
  "IW{1,1}(58,:)'" : Constant  Value=[-1.2435941564926358271492290441528894007205963134765625;0.696005022619397006877761668874882161617279052734375;-1.0303675349754881640507164775044657289981842041015625;-1.8115997633834515223583139231777749955654144287109375;0.9373981845036620796918214182369410991668701171875;2.28365113116096463130588745116256177425384521484375;-3.025956729824476720835946252918802201747894287109375;0.418683703383914196383130956746754236519336700439453125;0.143911923506624683799515196369611658155918121337890625]
      mask Display: e = 0.06;c1 = [120 150 230]/255;c2 = ([120 150 230]+0)/383;c3 = ([120 150 230]+128)/383;patch([0 1 1 0],[0 0 1 1],c1);patch([0 1 1 1-e 1-e 0+e],[0 0 1 1-e 0+e 0+e],c2);patch([0 0 1 1-e 0+e 0+e],[0 1 1 1-e 1-e 0+e],c3);plot([0 1 1 0 0],[0 0 1 1 0]);disp('Weights');
  "IW{1,1}(59,:)'" : Constant  Value=[-7.021119532831590959176537580788135528564453125;5.41686737457560330000205794931389391422271728515625;1.31969001776695282757145832874812185764312744140625;0.324437604839088289399029463311308063566684722900390625;-1.252802671194439998458847185247577726840972900390625;2.2203973761732669345292379148304462432861328125;1.13319943616672613728724172688089311122894287109375;-5.5808310233698108504540869034826755523681640625;3.32821771893894524652068866998888552188873291015625]
      mask Display: e = 0.06;c1 = [120 150 230]/255;c2 = ([120 150 230]+0)/383;c3 = ([120 150 230]+128)/383;patch([0 1 1 0],[0 0 1 1],c1);patch([0 1 1 1-e 1-e 0+e],[0 0 1 1-e 0+e 0+e],c2);patch([0 0 1 1-e 0+e 0+e],[0 1 1 1-e 1-e 0+e],c3);plot([0 1 1 0 0],[0 0 1 1 0]);disp('Weights');
  "IW{1,1}(6,:)'" : Constant  Value=[-3.477133037250531355510929643060080707073211669921875;5.536054595398557154339869157411158084869384765625;-4.3884973923132779560773997218348085880279541015625;-1.1185770130837282554381317822844721376895904541015625;1.194515231834520907483465634868480265140533447265625;0.2112717690901997069641282678276184014976024627685546875;4.021844283242909767750461469404399394989013671875;0.32709144720601657230218961558421142399311065673828125;-0.369118096303814535730225543375127017498016357421875]
      mask Display: e = 0.06;c1 = [120 150 230]/255;c2 = ([120 150 230]+0)/383;c3 = ([120 150 230]+128)/383;patch([0 1 1 0],[0 0 1 1],c1);patch([0 1 1 1-e 1-e 0+e],[0 0 1 1-e 0+e 0+e],c2);patch([0 0 1 1-e 0+e 0+e],[0 1 1 1-e 1-e 0+e],c3);plot([0 1 1 0 0],[0 0 1 1 0]);disp('Weights');
  "IW{1,1}(60,:)'" : Constant  Value=[2.07407629197529796982735206256620585918426513671875;-0.376382689697833894282297251265845261514186859130859375;4.1727888366341598924691425054334104061126708984375;0.2249948160940478392166852472655591554939746856689453125;-0.209457448471981833026944741504848934710025787353515625;0.12259035530817498360622863629032508470118045806884765625;-1.9885961569463888043429733443190343677997589111328125;-3.00546594661675925408417242579162120819091796875;1.016339325972172691336936622974462807178497314453125]
      mask Display: e = 0.06;c1 = [120 150 230]/255;c2 = ([120 150 230]+0)/383;c3 = ([120 150 230]+128)/383;patch([0 1 1 0],[0 0 1 1],c1);patch([0 1 1 1-e 1-e 0+e],[0 0 1 1-e 0+e 0+e],c2);patch([0 0 1 1-e 0+e 0+e],[0 1 1 1-e 1-e 0+e],c3);plot([0 1 1 0 0],[0 0 1 1 0]);disp('Weights');
  "IW{1,1}(61,:)'" : Constant  Value=[-0.319940379286479281706334631962818093597888946533203125;-1.267754567356095929397952204453758895397186279296875;1.3250367289308655482926724289427511394023895263671875;-1.04901555058556983368589499150402843952178955078125;-1.234822935931134679776732809841632843017578125;1.585207345821165514365702620125375688076019287109375;0.64227789578639626899558834338677115738391876220703125;1.6049668785723605335391539483680389821529388427734375;0.286632116496873090571995135178440250456333160400390625]
      mask Display: e = 0.06;c1 = [120 150 230]/255;c2 = ([120 150 230]+0)/383;c3 = ([120 150 230]+128)/383;patch([0 1 1 0],[0 0 1 1],c1);patch([0 1 1 1-e 1-e 0+e],[0 0 1 1-e 0+e 0+e],c2);patch([0 0 1 1-e 0+e 0+e],[0 1 1 1-e 1-e 0+e],c3);plot([0 1 1 0 0],[0 0 1 1 0]);disp('Weights');
  "IW{1,1}(62,:)'" : Constant  Value=[0.94618976807803989448331094536115415394306182861328125;0.38304565466729967315728799803764559328556060791015625;2.484424448671461949089689369429834187030792236328125;0.07791450826147851282943435080596827901899814605712890625;1.411822791781856434312203418812714517116546630859375;0.139349522213585874652608254109509289264678955078125;0.3208486702859507655460902242339216172695159912109375;1.2477582950142342976818099486990831792354583740234375;-0.03352017024961227720236678351284353993833065032958984375]
      mask Display: e = 0.06;c1 = [120 150 230]/255;c2 = ([120 150 230]+0)/383;c3 = ([120 150 230]+128)/383;patch([0 1 1 0],[0 0 1 1],c1);patch([0 1 1 1-e 1-e 0+e],[0 0 1 1-e 0+e 0+e],c2);patch([0 0 1 1-e 0+e 0+e],[0 1 1 1-e 1-e 0+e],c3);plot([0 1 1 0 0],[0 0 1 1 0]);disp('Weights');
  "IW{1,1}(63,:)'" : Constant  Value=[-1.83991842178087150472265420830808579921722412109375;1.811596235252487918643282682751305401325225830078125;-0.59161913426013101879874511723755858838558197021484375;0.62272595169897104749878735674428753554821014404296875;2.351464307400701780892404713085852563381195068359375;0.31381113483905942462826033079181797802448272705078125;0.99052934824598815044538469010149128735065460205078125;2.5860595832796864357305821613408625125885009765625;-0.0177123097157814886337678927930028294213116168975830078125]
      mask Display: e = 0.06;c1 = [120 150 230]/255;c2 = ([120 150 230]+0)/383;c3 = ([120 150 230]+128)/383;patch([0 1 1 0],[0 0 1 1],c1);patch([0 1 1 1-e 1-e 0+e],[0 0 1 1-e 0+e 0+e],c2);patch([0 0 1 1-e 0+e 0+e],[0 1 1 1-e 1-e 0+e],c3);plot([0 1 1 0 0],[0 0 1 1 0]);disp('Weights');
  "IW{1,1}(64,:)'" : Constant  Value=[-1.5762273654437322090160478182951919734477996826171875;-0.97321172787232035350513115190551616251468658447265625;0.39477878737687832622071937294094823300838470458984375;0.63092903590007110015136504443944431841373443603515625;-0.10119630106768322252985825571158784441649913787841796875;-1.087414188325173114435528987087309360504150390625;1.3988994401183429960866533292573876678943634033203125;-2.072294440301964524309141779667697846889495849609375;0.4354144379578175350076207905658520758152008056640625]
      mask Display: e = 0.06;c1 = [120 150 230]/255;c2 = ([120 150 230]+0)/383;c3 = ([120 150 230]+128)/383;patch([0 1 1 0],[0 0 1 1],c1);patch([0 1 1 1-e 1-e 0+e],[0 0 1 1-e 0+e 0+e],c2);patch([0 0 1 1-e 0+e 0+e],[0 1 1 1-e 1-e 0+e],c3);plot([0 1 1 0 0],[0 0 1 1 0]);disp('Weights');
  "IW{1,1}(65,:)'" : Constant  Value=[-0.81434473061368206625587617963901720941066741943359375;-2.186319763861188203435403920593671500682830810546875;0.84155508689486346884933709588949568569660186767578125;2.915901436696772375256614395766519010066986083984375;-0.0625448412503030459763664339334354735910892486572265625;2.4298889633398772502914653159677982330322265625;-1.18185277075212180619701030082069337368011474609375;-2.06836931495232168032316621975041925907135009765625;-2.2888859689998302116009654127992689609527587890625]
      mask Display: e = 0.06;c1 = [120 150 230]/255;c2 = ([120 150 230]+0)/383;c3 = ([120 150 230]+128)/383;patch([0 1 1 0],[0 0 1 1],c1);patch([0 1 1 1-e 1-e 0+e],[0 0 1 1-e 0+e 0+e],c2);patch([0 0 1 1-e 0+e 0+e],[0 1 1 1-e 1-e 0+e],c3);plot([0 1 1 0 0],[0 0 1 1 0]);disp('Weights');
  "IW{1,1}(66,:)'" : Constant  Value=[1.660598824284675867346550148795358836650848388671875;-1.3465689614926261707950061463634483516216278076171875;-5.0529013299743521514528765692375600337982177734375;-0.552193963717757529963137130835093557834625244140625;1.65600354457529430618478727410547435283660888671875;3.01278695139592667118222379940561950206756591796875;-2.586148588522323876759401173330843448638916015625;-0.5048506030494792629070843759109266102313995361328125;2.500503518951245229828828087192960083484649658203125]
      mask Display: e = 0.06;c1 = [120 150 230]/255;c2 = ([120 150 230]+0)/383;c3 = ([120 150 230]+128)/383;patch([0 1 1 0],[0 0 1 1],c1);patch([0 1 1 1-e 1-e 0+e],[0 0 1 1-e 0+e 0+e],c2);patch([0 0 1 1-e 0+e 0+e],[0 1 1 1-e 1-e 0+e],c3);plot([0 1 1 0 0],[0 0 1 1 0]);disp('Weights');
  "IW{1,1}(67,:)'" : Constant  Value=[3.59975319223486334152539711794815957546234130859375;-2.17609148817094411043626678292639553546905517578125;6.00242691217944202008993670460768043994903564453125;-1.1076723189558170812318849129951559007167816162109375;0.1122578196807179906624440945961396209895610809326171875;-0.31043023493415622393598596318042837083339691162109375;0.86254013587198752333051743335090577602386474609375;1.165749236231137242469912962405942380428314208984375;7.30481634479833186190944616100750863552093505859375]
      mask Display: e = 0.06;c1 = [120 150 230]/255;c2 = ([120 150 230]+0)/383;c3 = ([120 150 230]+128)/383;patch([0 1 1 0],[0 0 1 1],c1);patch([0 1 1 1-e 1-e 0+e],[0 0 1 1-e 0+e 0+e],c2);patch([0 0 1 1-e 0+e 0+e],[0 1 1 1-e 1-e 0+e],c3);plot([0 1 1 0 0],[0 0 1 1 0]);disp('Weights');
  "IW{1,1}(68,:)'" : Constant  Value=[6.897196162961744647645900840871036052703857421875;3.661527239085776930238580462173558771610260009765625;14.5290651690375991478276773705147206783294677734375;-1.7795545632925897638898504737881012260913848876953125;-0.70203729883363619190816962145618163049221038818359375;-1.5596066821405167868164198807789944112300872802734375;-0.7042594039136191863548219771473668515682220458984375;-4.1201483218043772893679488333873450756072998046875;-15.9052552729545677578926188289187848567962646484375]
      mask Display: e = 0.06;c1 = [120 150 230]/255;c2 = ([120 150 230]+0)/383;c3 = ([120 150 230]+128)/383;patch([0 1 1 0],[0 0 1 1],c1);patch([0 1 1 1-e 1-e 0+e],[0 0 1 1-e 0+e 0+e],c2);patch([0 0 1 1-e 0+e 0+e],[0 1 1 1-e 1-e 0+e],c3);plot([0 1 1 0 0],[0 0 1 1 0]);disp('Weights');
  "IW{1,1}(69,:)'" : Constant  Value=[-1.9801969671596719724249169303220696747303009033203125;1.9281149232037504415160356074920855462551116943359375;0.70235750389864037845910615942557342350482940673828125;0.72793443128612256298737293036538176238536834716796875;1.6940094887282064473055243070120923221111297607421875;1.718405651417847845863207112415693700313568115234375;-4.2029024676524837644819854176603257656097412109375;-0.342700129424788835219573002177639864385128021240234375;-2.532092852055703335878433790639974176883697509765625]
      mask Display: e = 0.06;c1 = [120 150 230]/255;c2 = ([120 150 230]+0)/383;c3 = ([120 150 230]+128)/383;patch([0 1 1 0],[0 0 1 1],c1);patch([0 1 1 1-e 1-e 0+e],[0 0 1 1-e 0+e 0+e],c2);patch([0 0 1 1-e 0+e 0+e],[0 1 1 1-e 1-e 0+e],c3);plot([0 1 1 0 0],[0 0 1 1 0]);disp('Weights');
  "IW{1,1}(7,:)'" : Constant  Value=[-2.57655777972624466798379216925241053104400634765625;4.389452966851788318081162287853658199310302734375;2.7689949662545387809586827643215656280517578125;0.75037080744514794705679605613113380968570709228515625;-1.9195897204510468103677567341946996748447418212890625;-0.5662589811757918756285334893618710339069366455078125;3.33958306712611285860248244716785848140716552734375;-5.419817469796125664061037241481244564056396484375;1.2482192998071262035608697260613553225994110107421875]
      mask Display: e = 0.06;c1 = [120 150 230]/255;c2 = ([120 150 230]+0)/383;c3 = ([120 150 230]+128)/383;patch([0 1 1 0],[0 0 1 1],c1);patch([0 1 1 1-e 1-e 0+e],[0 0 1 1-e 0+e 0+e],c2);patch([0 0 1 1-e 0+e 0+e],[0 1 1 1-e 1-e 0+e],c3);plot([0 1 1 0 0],[0 0 1 1 0]);disp('Weights');
  "IW{1,1}(70,:)'" : Constant  Value=[-2.221408378434948094337642032769508659839630126953125;-1.782973348276844394177942376700229942798614501953125;-3.729507408392321199386287844390608370304107666015625;-0.252992141664726888361514056668966077268123626708984375;5.34491704080483653882538419566117227077484130859375;-5.57093668854802448464624831103719770908355712890625;5.09076859653030400210127481841482222080230712890625;-2.362952745230430640077656789799220860004425048828125;1.4492497805540704991500433607143349945545196533203125]
      mask Display: e = 0.06;c1 = [120 150 230]/255;c2 = ([120 150 230]+0)/383;c3 = ([120 150 230]+128)/383;patch([0 1 1 0],[0 0 1 1],c1);patch([0 1 1 1-e 1-e 0+e],[0 0 1 1-e 0+e 0+e],c2);patch([0 0 1 1-e 0+e 0+e],[0 1 1 1-e 1-e 0+e],c3);plot([0 1 1 0 0],[0 0 1 1 0]);disp('Weights');
  "IW{1,1}(71,:)'" : Constant  Value=[-0.717213979650490163209042293601669371128082275390625;0.8516863682591593320836409475305117666721343994140625;-2.91837105772748284238105043186806142330169677734375;0.83205532861743558559197708746069110929965972900390625;-0.40403403561890571804582350523560307919979095458984375;-0.70823440825194350356497352549922652542591094970703125;-0.61007242499928115986307375351316295564174652099609375;-0.284660801869208446301939829936600290238857269287109375;0.2942550385295612525027308947755955159664154052734375]
      mask Display: e = 0.06;c1 = [120 150 230]/255;c2 = ([120 150 230]+0)/383;c3 = ([120 150 230]+128)/383;patch([0 1 1 0],[0 0 1 1],c1);patch([0 1 1 1-e 1-e 0+e],[0 0 1 1-e 0+e 0+e],c2);patch([0 0 1 1-e 0+e 0+e],[0 1 1 1-e 1-e 0+e],c3);plot([0 1 1 0 0],[0 0 1 1 0]);disp('Weights');
  "IW{1,1}(72,:)'" : Constant  Value=[1.4314165720177294272019707932486198842525482177734375;-3.2462389143752705678025449742563068866729736328125;1.7482086021259919395021142918267287313938140869140625;-0.08838599840138851304605083214482874609529972076416015625;2.45739549151791347725293235271237790584564208984375;-2.49104841531389720188371939002536237239837646484375;0.24989872963463788391180742110009305179119110107421875;-1.64354924758049225630429646116681396961212158203125;0.62965858083225978436558989415061660110950469970703125]
      mask Display: e = 0.06;c1 = [120 150 230]/255;c2 = ([120 150 230]+0)/383;c3 = ([120 150 230]+128)/383;patch([0 1 1 0],[0 0 1 1],c1);patch([0 1 1 1-e 1-e 0+e],[0 0 1 1-e 0+e 0+e],c2);patch([0 0 1 1-e 0+e 0+e],[0 1 1 1-e 1-e 0+e],c3);plot([0 1 1 0 0],[0 0 1 1 0]);disp('Weights');
  "IW{1,1}(73,:)'" : Constant  Value=[-0.78704102300655531809780995899927802383899688720703125;0.6412432997053105765417058137245476245880126953125;1.072056190820688481579736617277376353740692138671875;0.2240132848368218410062269185800687409937381744384765625;-0.07954811176887306711780212253870558924973011016845703125;0.83695015430473918005560562960454262793064117431640625;0.7804297293510067401456353763933293521404266357421875;1.988883760858371818613932191510684788227081298828125;-0.134237156335448581945257728875731118023395538330078125]
      mask Display: e = 0.06;c1 = [120 150 230]/255;c2 = ([120 150 230]+0)/383;c3 = ([120 150 230]+128)/383;patch([0 1 1 0],[0 0 1 1],c1);patch([0 1 1 1-e 1-e 0+e],[0 0 1 1-e 0+e 0+e],c2);patch([0 0 1 1-e 0+e 0+e],[0 1 1 1-e 1-e 0+e],c3);plot([0 1 1 0 0],[0 0 1 1 0]);disp('Weights');
  "IW{1,1}(74,:)'" : Constant  Value=[2.682123187087607885104034721734933555126190185546875;2.289398108416362820349831963540054857730865478515625;-0.91082144187935354384677566486061550676822662353515625;-2.272533776745932154739193720160983502864837646484375;1.3628617525478559091567376526654697954654693603515625;-2.0580814446986455124033454922027885913848876953125;0.29675556415049231251401806730427779257297515869140625;1.477960309655704573827961212373338639736175537109375;-0.58130659648126847827143137692473828792572021484375]
      mask Display: e = 0.06;c1 = [120 150 230]/255;c2 = ([120 150 230]+0)/383;c3 = ([120 150 230]+128)/383;patch([0 1 1 0],[0 0 1 1],c1);patch([0 1 1 1-e 1-e 0+e],[0 0 1 1-e 0+e 0+e],c2);patch([0 0 1 1-e 0+e 0+e],[0 1 1 1-e 1-e 0+e],c3);plot([0 1 1 0 0],[0 0 1 1 0]);disp('Weights');
  "IW{1,1}(75,:)'" : Constant  Value=[0.68010716662883885508250614293501712381839752197265625;1.3003775869360583161693512010970152914524078369140625;0.398352173947304155632309630163945257663726806640625;-0.177710782802932898416514717609970830380916595458984375;1.92148791458223744399447241448797285556793212890625;0.51991936233960267532694388137315399944782257080078125;6.264985568386396863616027985699474811553955078125;3.300858451008651162084106545080430805683135986328125;0.03239423805453985061308941340030287392437458038330078125]
      mask Display: e = 0.06;c1 = [120 150 230]/255;c2 = ([120 150 230]+0)/383;c3 = ([120 150 230]+128)/383;patch([0 1 1 0],[0 0 1 1],c1);patch([0 1 1 1-e 1-e 0+e],[0 0 1 1-e 0+e 0+e],c2);patch([0 0 1 1-e 0+e 0+e],[0 1 1 1-e 1-e 0+e],c3);plot([0 1 1 0 0],[0 0 1 1 0]);disp('Weights');
  "IW{1,1}(76,:)'" : Constant  Value=[1.01290877884510255313443849445320665836334228515625;-0.475572641500311699136460674708359874784946441650390625;-0.95375527389401437705629405172658152878284454345703125;0.4093717247055825847468213396496139466762542724609375;1.4816823266177345796990039161755703389644622802734375;0.50395681027192196221875519768218509852886199951171875;0.1527114765784302330420274529387825168669223785400390625;1.969468259302258328347079441300593316555023193359375;0.94236042200106784338942134127137251198291778564453125]
      mask Display: e = 0.06;c1 = [120 150 230]/255;c2 = ([120 150 230]+0)/383;c3 = ([120 150 230]+128)/383;patch([0 1 1 0],[0 0 1 1],c1);patch([0 1 1 1-e 1-e 0+e],[0 0 1 1-e 0+e 0+e],c2);patch([0 0 1 1-e 0+e 0+e],[0 1 1 1-e 1-e 0+e],c3);plot([0 1 1 0 0],[0 0 1 1 0]);disp('Weights');
  "IW{1,1}(77,:)'" : Constant  Value=[0.5189828882761065020901014577248133718967437744140625;0.378529876599773495993161986916675232350826263427734375;1.8275215299676517144433773864875547587871551513671875;1.3333520037153190340717401340953074395656585693359375;-2.62451239459922636143573981826193630695343017578125;-1.6208910006975905115922387267346493899822235107421875;-1.0546531875296369928918238656478933990001678466796875;-3.661398843751654919032034740666858851909637451171875;1.0256607822231718074590389733202755451202392578125]
      mask Display: e = 0.06;c1 = [120 150 230]/255;c2 = ([120 150 230]+0)/383;c3 = ([120 150 230]+128)/383;patch([0 1 1 0],[0 0 1 1],c1);patch([0 1 1 1-e 1-e 0+e],[0 0 1 1-e 0+e 0+e],c2);patch([0 0 1 1-e 0+e 0+e],[0 1 1 1-e 1-e 0+e],c3);plot([0 1 1 0 0],[0 0 1 1 0]);disp('Weights');
  "IW{1,1}(78,:)'" : Constant  Value=[-0.6719539152661380132514068463933654129505157470703125;0.0541820226436480478771073876487207598984241485595703125;0.55567530880328686038183150230906903743743896484375;1.6867984743108672684996918178512714803218841552734375;0.215937392800881922116928990362794138491153717041015625;1.3507287290250145073144949492416344583034515380859375;-0.09532239315981742844297031069800141267478466033935546875;0.4734420585682388438186762869008816778659820556640625;0.48337077203691813931385468094958923757076263427734375]
      mask Display: e = 0.06;c1 = [120 150 230]/255;c2 = ([120 150 230]+0)/383;c3 = ([120 150 230]+128)/383;patch([0 1 1 0],[0 0 1 1],c1);patch([0 1 1 1-e 1-e 0+e],[0 0 1 1-e 0+e 0+e],c2);patch([0 0 1 1-e 0+e 0+e],[0 1 1 1-e 1-e 0+e],c3);plot([0 1 1 0 0],[0 0 1 1 0]);disp('Weights');
  "IW{1,1}(79,:)'" : Constant  Value=[1.934157523113828158756177799659781157970428466796875;0.20267676130530409839280991945997811853885650634765625;0.85372965859497995655402746706386096775531768798828125;0.339085721556105834650907127070240676403045654296875;0.64264013898526151091772362633491866290569305419921875;1.5326937181080335648175605456344783306121826171875;1.007343797684885355891992730903439223766326904296875;-0.39607920088974746253285275088273920118808746337890625;-0.334634939272406672916559955410775728523731231689453125]
      mask Display: e = 0.06;c1 = [120 150 230]/255;c2 = ([120 150 230]+0)/383;c3 = ([120 150 230]+128)/383;patch([0 1 1 0],[0 0 1 1],c1);patch([0 1 1 1-e 1-e 0+e],[0 0 1 1-e 0+e 0+e],c2);patch([0 0 1 1-e 0+e 0+e],[0 1 1 1-e 1-e 0+e],c3);plot([0 1 1 0 0],[0 0 1 1 0]);disp('Weights');
  "IW{1,1}(8,:)'" : Constant  Value=[1.3272184533929263228202444224734790623188018798828125;0.54866455431879301851694208380649797618389129638671875;2.140180359974954260593449362204410135746002197265625;-0.2874703978403434501132096556830219924449920654296875;-1.2955370097399272477645126855350099503993988037109375;-1.352849956560000510563668285612948238849639892578125;1.607375688431591509441886955755762755870819091796875;1.2180885311930211845066196474363096058368682861328125;-0.8262862647117745762415097487973980605602264404296875]
      mask Display: e = 0.06;c1 = [120 150 230]/255;c2 = ([120 150 230]+0)/383;c3 = ([120 150 230]+128)/383;patch([0 1 1 0],[0 0 1 1],c1);patch([0 1 1 1-e 1-e 0+e],[0 0 1 1-e 0+e 0+e],c2);patch([0 0 1 1-e 0+e 0+e],[0 1 1 1-e 1-e 0+e],c3);plot([0 1 1 0 0],[0 0 1 1 0]);disp('Weights');
  "IW{1,1}(80,:)'" : Constant  Value=[1.569760157744060080631243181414902210235595703125;0.000301408942776177518098335017526778756291605532169342041015625;-1.8129968311668236413680688201566226780414581298828125;0.1302706067625724328795655537760467268526554107666015625;-0.41015300879845550952040866832248866558074951171875;1.4267665479585087684455402268213219940662384033203125;1.752955268603210381428425534977577626705169677734375;-0.2295884127115450923373174418884445913136005401611328125;-1.23488520152840219878953575971536338329315185546875]
      mask Display: e = 0.06;c1 = [120 150 230]/255;c2 = ([120 150 230]+0)/383;c3 = ([120 150 230]+128)/383;patch([0 1 1 0],[0 0 1 1],c1);patch([0 1 1 1-e 1-e 0+e],[0 0 1 1-e 0+e 0+e],c2);patch([0 0 1 1-e 0+e 0+e],[0 1 1 1-e 1-e 0+e],c3);plot([0 1 1 0 0],[0 0 1 1 0]);disp('Weights');
  "IW{1,1}(81,:)'" : Constant  Value=[2.756106066552046485185201163403689861297607421875;3.45104769532277710908374501741491258144378662109375;3.676842750777149060326109974994324147701263427734375;2.702784140548793789804449261282570660114288330078125;2.154250937667746779169419824029318988323211669921875;-0.428780904321171718596161781533737666904926300048828125;-1.3002879230373178831570157854002900421619415283203125;-0.145959090356595766468927877212991006672382354736328125;0.326208405082727637136486009694635868072509765625]
      mask Display: e = 0.06;c1 = [120 150 230]/255;c2 = ([120 150 230]+0)/383;c3 = ([120 150 230]+128)/383;patch([0 1 1 0],[0 0 1 1],c1);patch([0 1 1 1-e 1-e 0+e],[0 0 1 1-e 0+e 0+e],c2);patch([0 0 1 1-e 0+e 0+e],[0 1 1 1-e 1-e 0+e],c3);plot([0 1 1 0 0],[0 0 1 1 0]);disp('Weights');
  "IW{1,1}(82,:)'" : Constant  Value=[-1.4187105601741445415342468550079502165317535400390625;-2.406632670218321390365190381999127566814422607421875;-0.386278926046563164664604528297786600887775421142578125;-0.2350910083614413392805175817557028494775295257568359375;-0.24847857319674748755033988345530815422534942626953125;-1.872680959650208531996895544580183923244476318359375;0.5090511877944592367128961996058933436870574951171875;-0.422384781618223403842904417615500278770923614501953125;-1.3010143504796725100192134050303138792514801025390625]
      mask Display: e = 0.06;c1 = [120 150 230]/255;c2 = ([120 150 230]+0)/383;c3 = ([120 150 230]+128)/383;patch([0 1 1 0],[0 0 1 1],c1);patch([0 1 1 1-e 1-e 0+e],[0 0 1 1-e 0+e 0+e],c2);patch([0 0 1 1-e 0+e 0+e],[0 1 1 1-e 1-e 0+e],c3);plot([0 1 1 0 0],[0 0 1 1 0]);disp('Weights');
  "IW{1,1}(83,:)'" : Constant  Value=[-0.142384744211320413143084806506521999835968017578125;0.3649868965971754253274639268056489527225494384765625;-0.85611563815903368723780886284657754004001617431640625;1.3789848066088066236289932930958457291126251220703125;-0.1947824594137896603296411512928898446261882781982421875;1.709339957602454607155095800408162176609039306640625;0.99278963623935545523835344283725135028362274169921875;0.387072075840796170353996785706840455532073974609375;0.39010236195861214270053096697665750980377197265625]
      mask Display: e = 0.06;c1 = [120 150 230]/255;c2 = ([120 150 230]+0)/383;c3 = ([120 150 230]+128)/383;patch([0 1 1 0],[0 0 1 1],c1);patch([0 1 1 1-e 1-e 0+e],[0 0 1 1-e 0+e 0+e],c2);patch([0 0 1 1-e 0+e 0+e],[0 1 1 1-e 1-e 0+e],c3);plot([0 1 1 0 0],[0 0 1 1 0]);disp('Weights');
  "IW{1,1}(84,:)'" : Constant  Value=[0.34778184938683331939301979218726046383380889892578125;-0.71666728413282154708241478147101588547229766845703125;3.57733323454942375718701441655866801738739013671875;0.284859837422468398226982344567659310996532440185546875;0.30890627642410650732784915817319415509700775146484375;0.24158127647380245317521030301577411592006683349609375;1.991204024577047704269716632552444934844970703125;0.60790836831231553905041664620512165129184722900390625;-5.82931124336792105822269149939529597759246826171875]
      mask Display: e = 0.06;c1 = [120 150 230]/255;c2 = ([120 150 230]+0)/383;c3 = ([120 150 230]+128)/383;patch([0 1 1 0],[0 0 1 1],c1);patch([0 1 1 1-e 1-e 0+e],[0 0 1 1-e 0+e 0+e],c2);patch([0 0 1 1-e 0+e 0+e],[0 1 1 1-e 1-e 0+e],c3);plot([0 1 1 0 0],[0 0 1 1 0]);disp('Weights');
  "IW{1,1}(85,:)'" : Constant  Value=[0.156914420623106509733446500831632874906063079833984375;-0.24015056891083930157293480078806169331073760986328125;2.873357703146585340192586954799480736255645751953125;-0.515610710603976230004263925366103649139404296875;-0.412201059616510934180411140914657153189182281494140625;0.284689801343291082336151021081604994833469390869140625;0.402048396344202252361554883464123122394084930419921875;0.09646530617156699738412584110847092233598232269287109375;0.55679421899450165511780141969211399555206298828125]
      mask Display: e = 0.06;c1 = [120 150 230]/255;c2 = ([120 150 230]+0)/383;c3 = ([120 150 230]+128)/383;patch([0 1 1 0],[0 0 1 1],c1);patch([0 1 1 1-e 1-e 0+e],[0 0 1 1-e 0+e 0+e],c2);patch([0 0 1 1-e 0+e 0+e],[0 1 1 1-e 1-e 0+e],c3);plot([0 1 1 0 0],[0 0 1 1 0]);disp('Weights');
  "IW{1,1}(86,:)'" : Constant  Value=[-1.96202807078915508753880203585140407085418701171875;-10.31124036411761579756785067729651927947998046875;11.3246349140210345041168693569488823413848876953125;-3.7592758256182747800266952253878116607666015625;4.7901142718598404002250390476547181606292724609375;-0.60626181704465498256695354939438402652740478515625;1.8570568224666124113042542376206256449222564697265625;4.51003843967752349186639548861421644687652587890625;-5.7205909723562147206621375516988337039947509765625]
      mask Display: e = 0.06;c1 = [120 150 230]/255;c2 = ([120 150 230]+0)/383;c3 = ([120 150 230]+128)/383;patch([0 1 1 0],[0 0 1 1],c1);patch([0 1 1 1-e 1-e 0+e],[0 0 1 1-e 0+e 0+e],c2);patch([0 0 1 1-e 0+e 0+e],[0 1 1 1-e 1-e 0+e],c3);plot([0 1 1 0 0],[0 0 1 1 0]);disp('Weights');
  "IW{1,1}(87,:)'" : Constant  Value=[1.870779541276548219030928521533496677875518798828125;2.297862153948676766646030955598689615726470947265625;-2.42490609548104796289180740131996572017669677734375;-1.3668959758382419611422164962277747690677642822265625;-0.68239081329291462196806605788879096508026123046875;2.557633319021196172116106026805937290191650390625;-5.7973174110137346559668003465048968791961669921875;-0.9258811788763434691418297006748616695404052734375;0.7519144385695362142740805211360566318035125732421875]
      mask Display: e = 0.06;c1 = [120 150 230]/255;c2 = ([120 150 230]+0)/383;c3 = ([120 150 230]+128)/383;patch([0 1 1 0],[0 0 1 1],c1);patch([0 1 1 1-e 1-e 0+e],[0 0 1 1-e 0+e 0+e],c2);patch([0 0 1 1-e 0+e 0+e],[0 1 1 1-e 1-e 0+e],c3);plot([0 1 1 0 0],[0 0 1 1 0]);disp('Weights');
  "IW{1,1}(88,:)'" : Constant  Value=[-0.1068593241702182339292193091750959865748882293701171875;0.60931743433547314037213027404504828155040740966796875;0.9706493552256796331079158335342071950435638427734375;-0.19139289500859268944310542792663909494876861572265625;0.88964622229633516514724078660947270691394805908203125;1.0657600425787683295908436775789596140384674072265625;0.2923807553399953018669066295842640101909637451171875;1.0511338011636492950628962717019021511077880859375;-0.98495039306247722521447940380312502384185791015625]
      mask Display: e = 0.06;c1 = [120 150 230]/255;c2 = ([120 150 230]+0)/383;c3 = ([120 150 230]+128)/383;patch([0 1 1 0],[0 0 1 1],c1);patch([0 1 1 1-e 1-e 0+e],[0 0 1 1-e 0+e 0+e],c2);patch([0 0 1 1-e 0+e 0+e],[0 1 1 1-e 1-e 0+e],c3);plot([0 1 1 0 0],[0 0 1 1 0]);disp('Weights');
  "IW{1,1}(89,:)'" : Constant  Value=[-0.61196361540867905137730531350825913250446319580078125;-0.65014270660611150898233745465404354035854339599609375;1.745002506458528390709261657320894300937652587890625;0.313700871787627455500313544689561240375041961669921875;0.3817609348039521233175719316932372748851776123046875;0.55664523096122364709259500159532763063907623291015625;2.048200931144949610285266317077912390232086181640625;0.54817539009054050413993763868347741663455963134765625;-1.58549324797396540276395171531476080417633056640625]
      mask Display: e = 0.06;c1 = [120 150 230]/255;c2 = ([120 150 230]+0)/383;c3 = ([120 150 230]+128)/383;patch([0 1 1 0],[0 0 1 1],c1);patch([0 1 1 1-e 1-e 0+e],[0 0 1 1-e 0+e 0+e],c2);patch([0 0 1 1-e 0+e 0+e],[0 1 1 1-e 1-e 0+e],c3);plot([0 1 1 0 0],[0 0 1 1 0]);disp('Weights');
  "IW{1,1}(9,:)'" : Constant  Value=[-1.15925702564985311227019337820820510387420654296875;-0.043173147856086800666641778434495790861546993255615234375;1.331072485034713537288553197868168354034423828125;-1.7201446022824835591080727681401185691356658935546875;-0.288955869675199539248211522135534323751926422119140625;2.32476154576679849839138114475645124912261962890625;1.8400573237068924559167726329178549349308013916015625;1.2262473415571317758576697087846696376800537109375;-1.34790554551346275502510252408683300018310546875]
      mask Display: e = 0.06;c1 = [120 150 230]/255;c2 = ([120 150 230]+0)/383;c3 = ([120 150 230]+128)/383;patch([0 1 1 0],[0 0 1 1],c1);patch([0 1 1 1-e 1-e 0+e],[0 0 1 1-e 0+e 0+e],c2);patch([0 0 1 1-e 0+e 0+e],[0 1 1 1-e 1-e 0+e],c3);plot([0 1 1 0 0],[0 0 1 1 0]);disp('Weights');
  "IW{1,1}(90,:)'" : Constant  Value=[-1.0505475275797546697020834471913985908031463623046875;0.6733834006784624737207423095242120325565338134765625;0.561636916176877942774581242701970040798187255859375;1.467283368194749915147667707060463726520538330078125;-0.273837631244228718596644966964959166944026947021484375;-0.5704284717178016439476095911231823265552520751953125;-0.0102336569216798511927635217944043688476085662841796875;0.07706682868709945066765243382178596220910549163818359375;1.0038668642901871219663689771550707519054412841796875]
      mask Display: e = 0.06;c1 = [120 150 230]/255;c2 = ([120 150 230]+0)/383;c3 = ([120 150 230]+128)/383;patch([0 1 1 0],[0 0 1 1],c1);patch([0 1 1 1-e 1-e 0+e],[0 0 1 1-e 0+e 0+e],c2);patch([0 0 1 1-e 0+e 0+e],[0 1 1 1-e 1-e 0+e],c3);plot([0 1 1 0 0],[0 0 1 1 0]);disp('Weights');
  "IW{1,1}(91,:)'" : Constant  Value=[-1.65378395060932081861437836778350174427032470703125;4.51205878432818252576907980255782604217529296875;-1.0870949234777154135400678569567389786243438720703125;4.35897164463681985324683409999124705791473388671875;-0.08137930874002559378244114896006067283451557159423828125;-1.08184856109881177843590194243006408214569091796875;-0.0308313063275663969131645814059083932079374790191650390625;-3.90540606843474069620469890651293098926544189453125;3.682119573578742421915421800804324448108673095703125]
      mask Display: e = 0.06;c1 = [120 150 230]/255;c2 = ([120 150 230]+0)/383;c3 = ([120 150 230]+128)/383;patch([0 1 1 0],[0 0 1 1],c1);patch([0 1 1 1-e 1-e 0+e],[0 0 1 1-e 0+e 0+e],c2);patch([0 0 1 1-e 0+e 0+e],[0 1 1 1-e 1-e 0+e],c3);plot([0 1 1 0 0],[0 0 1 1 0]);disp('Weights');
  "IW{1,1}(92,:)'" : Constant  Value=[0.08846212397515317016338798339347704313695430755615234375;-4.6957434157599902135871161590330302715301513671875;-1.924831238000232591645044522010721266269683837890625;1.298414130481925443660884411656297743320465087890625;2.825299731605566133652018834254704415798187255859375;-4.5462718805079429529314438696019351482391357421875;-0.57674620361768258458567970592412166297435760498046875;2.879713981964071134456162326387129724025726318359375;0.299577178400173782524262833248940296471118927001953125]
      mask Display: e = 0.06;c1 = [120 150 230]/255;c2 = ([120 150 230]+0)/383;c3 = ([120 150 230]+128)/383;patch([0 1 1 0],[0 0 1 1],c1);patch([0 1 1 1-e 1-e 0+e],[0 0 1 1-e 0+e 0+e],c2);patch([0 0 1 1-e 0+e 0+e],[0 1 1 1-e 1-e 0+e],c3);plot([0 1 1 0 0],[0 0 1 1 0]);disp('Weights');
  "IW{1,1}(93,:)'" : Constant  Value=[-0.60863142594671926222105184933752752840518951416015625;0.608451515616527327523499479866586625576019287109375;-0.5894816610498445630383912430261261761188507080078125;0.0540476782785350440274640959614771418273448944091796875;2.08406973357340774555268581025302410125732421875;-1.9054268782855519059893367739277891814708709716796875;1.35874915004356910941396563430316746234893798828125;-0.395661678468714417267193539373693056404590606689453125;-1.2555150091124780420415163462166674435138702392578125]
      mask Display: e = 0.06;c1 = [120 150 230]/255;c2 = ([120 150 230]+0)/383;c3 = ([120 150 230]+128)/383;patch([0 1 1 0],[0 0 1 1],c1);patch([0 1 1 1-e 1-e 0+e],[0 0 1 1-e 0+e 0+e],c2);patch([0 0 1 1-e 0+e 0+e],[0 1 1 1-e 1-e 0+e],c3);plot([0 1 1 0 0],[0 0 1 1 0]);disp('Weights');
  "IW{1,1}(94,:)'" : Constant  Value=[-4.6718016724134283634839448495768010616302490234375;5.119823865480416458240142674185335636138916015625;-15.648389673288807699691460584290325641632080078125;-0.79727395750004126373511326164589263498783111572265625;3.111485680595833525075022407690994441509246826171875;1.34521045675742101366267888806760311126708984375;-2.0528627808095851747793858521617949008941650390625;3.871451508269864394407022700761444866657257080078125;0.88755049722952705781864324308116920292377471923828125]
      mask Display: e = 0.06;c1 = [120 150 230]/255;c2 = ([120 150 230]+0)/383;c3 = ([120 150 230]+128)/383;patch([0 1 1 0],[0 0 1 1],c1);patch([0 1 1 1-e 1-e 0+e],[0 0 1 1-e 0+e 0+e],c2);patch([0 0 1 1-e 0+e 0+e],[0 1 1 1-e 1-e 0+e],c3);plot([0 1 1 0 0],[0 0 1 1 0]);disp('Weights');
  "IW{1,1}(95,:)'" : Constant  Value=[-0.2128952617425768634173977034151903353631496429443359375;0.6856060824368928052763294545002281665802001953125;0.96690346082123002080521700918325223028659820556640625;0.50640182719382220710713227163068950176239013671875;0.73952795647169067283499543918878771364688873291015625;0.60241955816290493341824685558094643056392669677734375;1.125103732255608779411204523057676851749420166015625;-0.79041994784177715960282739615649916231632232666015625;0.96225346917812626390542618537438102066516876220703125]
      mask Display: e = 0.06;c1 = [120 150 230]/255;c2 = ([120 150 230]+0)/383;c3 = ([120 150 230]+128)/383;patch([0 1 1 0],[0 0 1 1],c1);patch([0 1 1 1-e 1-e 0+e],[0 0 1 1-e 0+e 0+e],c2);patch([0 0 1 1-e 0+e 0+e],[0 1 1 1-e 1-e 0+e],c3);plot([0 1 1 0 0],[0 0 1 1 0]);disp('Weights');
  "IW{1,1}(96,:)'" : Constant  Value=[1.0967346416990702007154823149903677403926849365234375;0.922566504700147671513832392520271241664886474609375;-0.1636071160624026077368142750856350176036357879638671875;1.691394792946223191165699972771108150482177734375;-2.22537684681821001930757120135240256786346435546875;-0.70287040902730713032298126563546247780323028564453125;1.4460713691449400553068471708684228360652923583984375;-1.1684231404524505482100948938750661909580230712890625;-1.2582975244287553096000920049846172332763671875]
      mask Display: e = 0.06;c1 = [120 150 230]/255;c2 = ([120 150 230]+0)/383;c3 = ([120 150 230]+128)/383;patch([0 1 1 0],[0 0 1 1],c1);patch([0 1 1 1-e 1-e 0+e],[0 0 1 1-e 0+e 0+e],c2);patch([0 0 1 1-e 0+e 0+e],[0 1 1 1-e 1-e 0+e],c3);plot([0 1 1 0 0],[0 0 1 1 0]);disp('Weights');
  "IW{1,1}(97,:)'" : Constant  Value=[-0.1688348251256373000472876810817979276180267333984375;0.39163336811279225724291563892620615661144256591796875;0.92656864868625954390068955035530962049961090087890625;0.72548216542411003704415861648158170282840728759765625;0.86107652071232287926960680124466307461261749267578125;-1.1429490156330734951239946894929744303226470947265625;-0.352677043424857117326354227770934812724590301513671875;0.98221873419602967469899112984421662986278533935546875;0.84384093814381599951701673489878885447978973388671875]
      mask Display: e = 0.06;c1 = [120 150 230]/255;c2 = ([120 150 230]+0)/383;c3 = ([120 150 230]+128)/383;patch([0 1 1 0],[0 0 1 1],c1);patch([0 1 1 1-e 1-e 0+e],[0 0 1 1-e 0+e 0+e],c2);patch([0 0 1 1-e 0+e 0+e],[0 1 1 1-e 1-e 0+e],c3);plot([0 1 1 0 0],[0 0 1 1 0]);disp('Weights');
  "IW{1,1}(98,:)'" : Constant  Value=[-4.1379997458992843206715406267903745174407958984375;-0.125416012282852984416336994399898685514926910400390625;4.46979373938678303801452784682624042034149169921875;3.375511262845673154942005567136220633983612060546875;-0.99712099096010164966941147213219664990901947021484375;-4.88001910121547322063406681991182267665863037109375;-0.67367762206182835171830447507090866565704345703125;4.4617133752831232840208031120710074901580810546875;1.903716645476388524826916182064451277256011962890625]
      mask Display: e = 0.06;c1 = [120 150 230]/255;c2 = ([120 150 230]+0)/383;c3 = ([120 150 230]+128)/383;patch([0 1 1 0],[0 0 1 1],c1);patch([0 1 1 1-e 1-e 0+e],[0 0 1 1-e 0+e 0+e],c2);patch([0 0 1 1-e 0+e 0+e],[0 1 1 1-e 1-e 0+e],c3);plot([0 1 1 0 0],[0 0 1 1 0]);disp('Weights');
  "IW{1,1}(99,:)'" : Constant  Value=[-0.653124246361963312068610321148298680782318115234375;0.01239129907538414308854068934806491597555577754974365234375;-0.53755339020441261776994679166818968951702117919921875;-1.21741851274706558427851632586680352687835693359375;-0.204380100272171072450788642527186311781406402587890625;0.41781131639760504814518071725615300238132476806640625;-2.72552080749518399471753582474775612354278564453125;1.38135886431515420014193296083249151706695556640625;0.826893859195525049443631360190920531749725341796875]
      mask Display: e = 0.06;c1 = [120 150 230]/255;c2 = ([120 150 230]+0)/383;c3 = ([120 150 230]+128)/383;patch([0 1 1 0],[0 0 1 1],c1);patch([0 1 1 1-e 1-e 0+e],[0 0 1 1-e 0+e 0+e],c2);patch([0 0 1 1-e 0+e 0+e],[0 1 1 1-e 1-e 0+e],c3);plot([0 1 1 0 0],[0 0 1 1 0]);disp('Weights');
  Mux : Mux  Inputs=100
      mask Display: e = 0.06;c1 = [120 150 230]/255;c2 = ([120 150 230]+0)/383;c3 = ([120 150 230]+128)/383;patch([0 1 1 0],[0 0 1 1],c1);patch([0 1 1 1-e 1-e 0+e],[0 0 1 1-e 0+e 0+e],c2);patch([0 0 1 1-e 0+e 0+e],[0 1 1 1-e 1-e 0+e],c3);plot([0 1 1 0 0],[0 0 1 1 0]);disp('Mux');
  dotprod{1..100} (100 alike) : neural/Weight Functions/dotprod
  "iz{1,1}" : Outport
      mask Display: e = 0.06;c1 = [120 230 180]/255;c2 = ([120 230 180]+0)/(256+128);c3 = ([120 230 180]+128)/(256+128);patch([0 1 1 0],[0 0 1 1],c1);patch([0 1 1 1-e 1-e 0+e],[0 0 1 1-e 0+e 0+e],c2);patch([0 0 1 1-e 0+e 0+e],[0 1 1 1-e 1-e 0+e],c3);plot([0 1 1 0 0],[0 0 1 1 0]);
  wires:
  "IW{1,1}(1,:)'"/1 -> dotprod1/1
  "pd{1,1}"/1 -> dotprod1/2, dotprod2/2, dotprod3/2, dotprod4/2, dotprod5/2, dotprod6/2, dotprod7/2, dotprod8/2, dotprod9/2, dotprod10/2, dotprod11/2, dotprod12/2, dotprod13/2, dotprod14/2, dotprod15/2, dotprod16/2, dotprod17/2, dotprod18/2, dotprod19/2, dotprod20/2, dotprod21/2, dotprod22/2, dotprod23/2, dotprod24/2, dotprod25/2, dotprod26/2, dotprod27/2, dotprod28/2, dotprod29/2, dotprod30/2, dotprod31/2, dotprod32/2, dotprod33/2, dotprod34/2, dotprod35/2, dotprod36/2, dotprod37/2, dotprod38/2, dotprod39/2, dotprod40/2, dotprod41/2, dotprod42/2, dotprod43/2, dotprod44/2, dotprod45/2, dotprod46/2, dotprod47/2, dotprod48/2, dotprod49/2, dotprod50/2, dotprod51/2, dotprod52/2, dotprod53/2, dotprod54/2, dotprod55/2, dotprod56/2, dotprod57/2, dotprod58/2, dotprod59/2, dotprod60/2, dotprod61/2, dotprod62/2, dotprod63/2, dotprod64/2, dotprod65/2, dotprod66/2, dotprod67/2, dotprod68/2, dotprod69/2, dotprod70/2, dotprod71/2, dotprod72/2, dotprod73/2, dotprod74/2, dotprod75/2, dotprod76/2, dotprod77/2, dotprod78/2, dotprod79/2, dotprod80/2, dotprod81/2, dotprod82/2, dotprod83/2, dotprod84/2, dotprod85/2, dotprod86/2, dotprod87/2, dotprod88/2, dotprod89/2, dotprod90/2, dotprod91/2, dotprod92/2, dotprod93/2, dotprod94/2, dotprod95/2, dotprod96/2, dotprod97/2, dotprod98/2, dotprod99/2, dotprod100/2
  dotprod1/1 -> Mux/1
  "IW{1,1}(2,:)'"/1 -> dotprod2/1
  dotprod2/1 -> Mux/2
  "IW{1,1}(3,:)'"/1 -> dotprod3/1
  dotprod3/1 -> Mux/3
  "IW{1,1}(4,:)'"/1 -> dotprod4/1
  dotprod4/1 -> Mux/4
  "IW{1,1}(5,:)'"/1 -> dotprod5/1
  dotprod5/1 -> Mux/5
  "IW{1,1}(6,:)'"/1 -> dotprod6/1
  dotprod6/1 -> Mux/6
  "IW{1,1}(7,:)'"/1 -> dotprod7/1
  dotprod7/1 -> Mux/7
  "IW{1,1}(8,:)'"/1 -> dotprod8/1
  dotprod8/1 -> Mux/8
  "IW{1,1}(9,:)'"/1 -> dotprod9/1
  dotprod9/1 -> Mux/9
  "IW{1,1}(10,:)'"/1 -> dotprod10/1
  dotprod10/1 -> Mux/10
  "IW{1,1}(11,:)'"/1 -> dotprod11/1
  dotprod11/1 -> Mux/11
  "IW{1,1}(12,:)'"/1 -> dotprod12/1
  dotprod12/1 -> Mux/12
  "IW{1,1}(13,:)'"/1 -> dotprod13/1
  dotprod13/1 -> Mux/13
  "IW{1,1}(14,:)'"/1 -> dotprod14/1
  dotprod14/1 -> Mux/14
  "IW{1,1}(15,:)'"/1 -> dotprod15/1
  dotprod15/1 -> Mux/15
  "IW{1,1}(16,:)'"/1 -> dotprod16/1
  dotprod16/1 -> Mux/16
  "IW{1,1}(17,:)'"/1 -> dotprod17/1
  dotprod17/1 -> Mux/17
  "IW{1,1}(18,:)'"/1 -> dotprod18/1
  dotprod18/1 -> Mux/18
  "IW{1,1}(19,:)'"/1 -> dotprod19/1
  dotprod19/1 -> Mux/19
  "IW{1,1}(20,:)'"/1 -> dotprod20/1
  dotprod20/1 -> Mux/20
  "IW{1,1}(21,:)'"/1 -> dotprod21/1
  dotprod21/1 -> Mux/21
  "IW{1,1}(22,:)'"/1 -> dotprod22/1
  dotprod22/1 -> Mux/22
  "IW{1,1}(23,:)'"/1 -> dotprod23/1
  dotprod23/1 -> Mux/23
  "IW{1,1}(24,:)'"/1 -> dotprod24/1
  dotprod24/1 -> Mux/24
  "IW{1,1}(25,:)'"/1 -> dotprod25/1
  dotprod25/1 -> Mux/25
  "IW{1,1}(26,:)'"/1 -> dotprod26/1
  dotprod26/1 -> Mux/26
  "IW{1,1}(27,:)'"/1 -> dotprod27/1
  dotprod27/1 -> Mux/27
  "IW{1,1}(28,:)'"/1 -> dotprod28/1
  dotprod28/1 -> Mux/28
  "IW{1,1}(29,:)'"/1 -> dotprod29/1
  dotprod29/1 -> Mux/29
  "IW{1,1}(30,:)'"/1 -> dotprod30/1
  dotprod30/1 -> Mux/30
  "IW{1,1}(31,:)'"/1 -> dotprod31/1
  dotprod31/1 -> Mux/31
  "IW{1,1}(32,:)'"/1 -> dotprod32/1
  dotprod32/1 -> Mux/32
  "IW{1,1}(33,:)'"/1 -> dotprod33/1
  dotprod33/1 -> Mux/33
  "IW{1,1}(34,:)'"/1 -> dotprod34/1
  dotprod34/1 -> Mux/34
  "IW{1,1}(35,:)'"/1 -> dotprod35/1
  dotprod35/1 -> Mux/35
  "IW{1,1}(36,:)'"/1 -> dotprod36/1
  dotprod36/1 -> Mux/36
  "IW{1,1}(37,:)'"/1 -> dotprod37/1
  dotprod37/1 -> Mux/37
  "IW{1,1}(38,:)'"/1 -> dotprod38/1
  dotprod38/1 -> Mux/38
  "IW{1,1}(39,:)'"/1 -> dotprod39/1
  dotprod39/1 -> Mux/39
  "IW{1,1}(40,:)'"/1 -> dotprod40/1
  dotprod40/1 -> Mux/40
  "IW{1,1}(41,:)'"/1 -> dotprod41/1
  dotprod41/1 -> Mux/41
  "IW{1,1}(42,:)'"/1 -> dotprod42/1
  dotprod42/1 -> Mux/42
  "IW{1,1}(43,:)'"/1 -> dotprod43/1
  dotprod43/1 -> Mux/43
  "IW{1,1}(44,:)'"/1 -> dotprod44/1
  dotprod44/1 -> Mux/44
  "IW{1,1}(45,:)'"/1 -> dotprod45/1
  dotprod45/1 -> Mux/45
  "IW{1,1}(46,:)'"/1 -> dotprod46/1
  dotprod46/1 -> Mux/46
  "IW{1,1}(47,:)'"/1 -> dotprod47/1
  dotprod47/1 -> Mux/47
  "IW{1,1}(48,:)'"/1 -> dotprod48/1
  dotprod48/1 -> Mux/48
  "IW{1,1}(49,:)'"/1 -> dotprod49/1
  dotprod49/1 -> Mux/49
  "IW{1,1}(50,:)'"/1 -> dotprod50/1
  dotprod50/1 -> Mux/50
  "IW{1,1}(51,:)'"/1 -> dotprod51/1
  dotprod51/1 -> Mux/51
  "IW{1,1}(52,:)'"/1 -> dotprod52/1
  dotprod52/1 -> Mux/52
  "IW{1,1}(53,:)'"/1 -> dotprod53/1
  dotprod53/1 -> Mux/53
  "IW{1,1}(54,:)'"/1 -> dotprod54/1
  dotprod54/1 -> Mux/54
  "IW{1,1}(55,:)'"/1 -> dotprod55/1
  dotprod55/1 -> Mux/55
  "IW{1,1}(56,:)'"/1 -> dotprod56/1
  dotprod56/1 -> Mux/56
  "IW{1,1}(57,:)'"/1 -> dotprod57/1
  dotprod57/1 -> Mux/57
  "IW{1,1}(58,:)'"/1 -> dotprod58/1
  dotprod58/1 -> Mux/58
  "IW{1,1}(59,:)'"/1 -> dotprod59/1
  dotprod59/1 -> Mux/59
  "IW{1,1}(60,:)'"/1 -> dotprod60/1
  dotprod60/1 -> Mux/60
  "IW{1,1}(61,:)'"/1 -> dotprod61/1
  dotprod61/1 -> Mux/61
  "IW{1,1}(62,:)'"/1 -> dotprod62/1
  dotprod62/1 -> Mux/62
  "IW{1,1}(63,:)'"/1 -> dotprod63/1
  dotprod63/1 -> Mux/63
  "IW{1,1}(64,:)'"/1 -> dotprod64/1
  dotprod64/1 -> Mux/64
  "IW{1,1}(65,:)'"/1 -> dotprod65/1
  dotprod65/1 -> Mux/65
  "IW{1,1}(66,:)'"/1 -> dotprod66/1
  dotprod66/1 -> Mux/66
  "IW{1,1}(67,:)'"/1 -> dotprod67/1
  dotprod67/1 -> Mux/67
  "IW{1,1}(68,:)'"/1 -> dotprod68/1
  dotprod68/1 -> Mux/68
  "IW{1,1}(69,:)'"/1 -> dotprod69/1
  dotprod69/1 -> Mux/69
  "IW{1,1}(70,:)'"/1 -> dotprod70/1
  dotprod70/1 -> Mux/70
  "IW{1,1}(71,:)'"/1 -> dotprod71/1
  dotprod71/1 -> Mux/71
  "IW{1,1}(72,:)'"/1 -> dotprod72/1
  dotprod72/1 -> Mux/72
  "IW{1,1}(73,:)'"/1 -> dotprod73/1
  dotprod73/1 -> Mux/73
  "IW{1,1}(74,:)'"/1 -> dotprod74/1
  dotprod74/1 -> Mux/74
  "IW{1,1}(75,:)'"/1 -> dotprod75/1
  dotprod75/1 -> Mux/75
  "IW{1,1}(76,:)'"/1 -> dotprod76/1
  dotprod76/1 -> Mux/76
  "IW{1,1}(77,:)'"/1 -> dotprod77/1
  dotprod77/1 -> Mux/77
  "IW{1,1}(78,:)'"/1 -> dotprod78/1
  dotprod78/1 -> Mux/78
  "IW{1,1}(79,:)'"/1 -> dotprod79/1
  dotprod79/1 -> Mux/79
  "IW{1,1}(80,:)'"/1 -> dotprod80/1
  dotprod80/1 -> Mux/80
  "IW{1,1}(81,:)'"/1 -> dotprod81/1
  dotprod81/1 -> Mux/81
  "IW{1,1}(82,:)'"/1 -> dotprod82/1
  dotprod82/1 -> Mux/82
  "IW{1,1}(83,:)'"/1 -> dotprod83/1
  dotprod83/1 -> Mux/83
  "IW{1,1}(84,:)'"/1 -> dotprod84/1
  dotprod84/1 -> Mux/84
  "IW{1,1}(85,:)'"/1 -> dotprod85/1
  dotprod85/1 -> Mux/85
  "IW{1,1}(86,:)'"/1 -> dotprod86/1
  dotprod86/1 -> Mux/86
  "IW{1,1}(87,:)'"/1 -> dotprod87/1
  dotprod87/1 -> Mux/87
  "IW{1,1}(88,:)'"/1 -> dotprod88/1
  dotprod88/1 -> Mux/88
  "IW{1,1}(89,:)'"/1 -> dotprod89/1
  dotprod89/1 -> Mux/89
  "IW{1,1}(90,:)'"/1 -> dotprod90/1
  dotprod90/1 -> Mux/90
  "IW{1,1}(91,:)'"/1 -> dotprod91/1
  dotprod91/1 -> Mux/91
  "IW{1,1}(92,:)'"/1 -> dotprod92/1
  dotprod92/1 -> Mux/92
  "IW{1,1}(93,:)'"/1 -> dotprod93/1
  dotprod93/1 -> Mux/93
  "IW{1,1}(94,:)'"/1 -> dotprod94/1
  dotprod94/1 -> Mux/94
  "IW{1,1}(95,:)'"/1 -> dotprod95/1
  dotprod95/1 -> Mux/95
  "IW{1,1}(96,:)'"/1 -> dotprod96/1
  dotprod96/1 -> Mux/96
  "IW{1,1}(97,:)'"/1 -> dotprod97/1
  dotprod97/1 -> Mux/97
  "IW{1,1}(98,:)'"/1 -> dotprod98/1
  dotprod98/1 -> Mux/98
  "IW{1,1}(99,:)'"/1 -> dotprod99/1
  dotprod99/1 -> Mux/99
  "IW{1,1}(100,:)'"/1 -> dotprod100/1
  dotprod100/1 -> Mux/100
  Mux/1 -> "iz{1,1}"/1
